simulink model "finalmodel1"  (R2024b)
(part 5 of 9)

POWER CORP D6P285A4F | NEO SOLAR POWER CORP D6P285A4FME | NEO SOLAR POWER CORP D6P285B4A | NEO SOLAR POWER CORP D6P285B4AME | NEO SOLAR POWER CORP D6Q285B4A | NEO SOLAR POWER CORP D6Q285B4AME | NEO SOLAR POWER CORP 7C00-6C290 | NEO SOLAR POWER CORP 7C00-6C290-B | NEO SOLAR POWER CORP 7E00-6C290 | NEO SOLAR POWER CORP 7E00-6C290-B | NEO SOLAR POWER CORP D6M290B3A | NEO SOLAR POWER CORP D6M290B3AME | NEO SOLAR POWER CORP D6M290B4A | NEO SOLAR POWER CORP D6M290B4AME | NEO SOLAR POWER CORP D6M290E3A | NEO SOLAR POWER CORP D6M290H3A | NEO SOLAR POWER CORP D6P290A4F | NEO SOLAR POWER CORP D6P290A4FME | NEO SOLAR POWER CORP D6P290B4A | NEO SOLAR POWER CORP D6P290B4AME | NEO SOLAR POWER CORP D6Q290B4A | NEO SOLAR POWER CORP D6Q290B4AME | NEO SOLAR POWER CORP 7C00-6C295 | NEO SOLAR POWER CORP 7C00-6C295-B | NEO SOLAR POWER CORP 7E00-6C295 | NEO SOLAR POWER CORP 7E00-6C295-B | NEO SOLAR POWER CORP D6M295B3A | NEO SOLAR POWER CORP D6M295B3AME | NEO SOLAR POWER CORP D6M295B4A | NEO SOLAR POWER CORP D6M295B4AME | NEO SOLAR POWER CORP D6M295E3A | NEO SOLAR POWER CORP D6M295H3A | NEO SOLAR POWER CORP D6P295B4A | NEO SOLAR POWER CORP D6P295B4AME | NEO SOLAR POWER CORP D6Q295B4A | NEO SOLAR POWER CORP D6Q295B4AME | NEO SOLAR POWER CORP 7E00-6C300 | NEO SOLAR POWER CORP 7E00-6C300-B | NEO SOLAR POWER CORP D6M300B3A | NEO SOLAR POWER CORP D6M300B3AME | NEO SOLAR POWER CORP D6M300B4A | NEO SOLAR POWER CORP D6M300B4AME | NEO SOLAR POWER CORP D6M300E3A | NEO SOLAR POWER CORP D6M300H3A | NEO SOLAR POWER CORP D6P300B4A | NEO SOLAR POWER CORP D6P300B4AME | NEO SOLAR POWER CORP 7E00-6C305 | NEO SOLAR POWER CORP 7E00-6C305-B | NEO SOLAR POWER CORP D6M305B4A | NEO SOLAR POWER CORP D6M305B4AME | NEO SOLAR POWER CORP D6M305E3A | NEO SOLAR POWER CORP D6M305H3A | NEO SOLAR POWER CORP D6P305B4A | NEO SOLAR POWER CORP D6P305B4AME | NEO SOLAR POWER CORP D6M310B4A | NEO SOLAR POWER CORP D6M310B4AME | NEO SOLAR POWER CORP D6M310E3A | NEO SOLAR POWER CORP D6M310H3A | NEO SOLAR POWER CORP D6P310B4A | NEO SOLAR POWER CORP D6P310B4AME | NEO SOLAR POWER CORP D6M315B4A | NEO SOLAR POWER CORP D6M315B4AME | NEO SOLAR POWER CORP D6M315E4A | NEO SOLAR POWER CORP D6M315E4AME | NEO SOLAR POWER CORP D6M315H3A | NEO SOLAR POWER CORP D6P315B4A | NEO SOLAR POWER CORP D6P315B4AME | NEO SOLAR POWER CORP D6M320B4A | NEO SOLAR POWER CORP D6M320B4AME | NEO SOLAR POWER CORP D6M320E4A | NEO SOLAR POWER CORP D6M320E4AME | NEO SOLAR POWER CORP D6M320H3A | NEO SOLAR POWER CORP D6P320B4A | NEO SOLAR POWER CORP D6P320B4AME | NEO SOLAR POWER CORP D6M325B4A | NEO SOLAR POWER CORP D6M325B4AME | NEO SOLAR POWER CORP D6M325E4A | NEO SOLAR POWER CORP D6M325E4AME | NEO SOLAR POWER CORP D6M325H3A | NEO SOLAR POWER CORP D6P325B4A | NEO SOLAR POWER CORP D6P325B4AME | NEO SOLAR POWER CORP D6M330B4A | NEO SOLAR POWER CORP D6M330B4AME | NEO SOLAR POWER CORP D6M330E4A | NEO SOLAR POWER CORP D6M330E4AME | NEO SOLAR POWER CORP D6M330H4A | NEO SOLAR POWER CORP D6P330B4A | NEO SOLAR POWER CORP D6P330B4AME | NEO SOLAR POWER CORP D6M335B4A | NEO SOLAR POWER CORP D6M335B4AME | NEO SOLAR POWER CORP D6M335E4A | NEO SOLAR POWER CORP D6M335E4AME | NEO SOLAR POWER CORP D6M335H4A | NEO SOLAR POWER CORP D6M340E4A | NEO SOLAR POWER CORP D6M340E4AME | NEO SOLAR POWER CORP D6M340H4A | NEO SOLAR POWER CORP D6M345E4A | NEO SOLAR POWER CORP D6M345E4AME | NEO SOLAR POWER CORP D6M345H4A | NEO SOLAR POWER CORP D6M350E4A | NEO SOLAR POWER CORP D6M350E4AME | NEO SOLAR POWER CORP D6M350H4A | NEO SOLAR POWER CORP D6M355E4A | NEO SOLAR POWER CORP D6M355E4AME | NEO SOLAR POWER CORP D6M355H4A | NEO SOLAR POWER CORP D6M360E4A | NEO SOLAR POWER CORP D6M360E4AME | NEO SOLAR POWER CORP D6M360H4A | NEO SOLAR POWER CORP D6M365E4A | NEO SOLAR POWER CORP D6M365E4AME | NEO SOLAR POWER CORP D6M365H4A | NEO SOLAR POWER CORP D6M370E4A | NEO SOLAR POWER CORP D6M370E4AME | NEO SOLAR POWER CORP D6M370H4A | NEO SOLAR POWER CORP D6M375E4A | NEO SOLAR POWER CORP D6M375E4AME | NEO SOLAR POWER CORP D6M375H4A | NEO SOLAR POWER CORP D6M380E4A | NEO SOLAR POWER CORP D6M380E4AME | NEO SOLAR POWER CORP D6M380H4A | NexPower Technology NH-100UT_3A | NexPower Technology NH-100UX 3A | NexPower Technology NH-100UT_4A | NexPower Technology NH-100UX 4A | NexPower Technology NH-100UT_5A | NexPower Technology NH-100UX 5A | NexPower Technology NH-100UT_6A | NexPower Technology NT-125UX | NexPower Technology NT-130UX | NexPower Technology NT-135UX | NexPower Technology NT-140UX | NexPower Technology NT-145UX | NexPower Technology NT-150 | NexPower Technology NT-155 | Next Solar Systems NXT18m | Next Solar Systems NXT20e | NICOR NS-H115M54-01 | NICOR NS-H120M54-01 | NICOR NS-H125M54-01 | NICOR NS-H160M72-01 | NICOR NS-H165M72-01 | NICOR NS-H170M72-01 | NICOR NS-H175M72-01 | NICOR NS-H180M72-01 | NICOR NS-H185M72-01 | NICOR NS-H190M72-01 | NICOR NS-H195M72-01 | NICOR NS-H200M72-01 | NICOR NS-H200P60-01 | NICOR NS-H205P60-01 | NICOR NS-H210P60-01 | NICOR NS-H215P60-01 | NICOR NS-H220P60-01 | NICOR NS-H225P60-01 | NICOR NS-H230P60-01 | NICOR NS-H235P60-01 | NICOR NS-H240P60-01 | Ningbo Best Solar Energy Technology B155(35)P1580X800 | Ningbo Best Solar Energy Technology B160(35)P1580X800 | Ningbo Best Solar Energy Technology B165(35)P1580X800 | Ningbo Best Solar Energy Technology B175(35)P1580X800 | Ningbo Best Solar Energy Technology B180(35)P1580X800 | Ningbo Maxsolar MP-150WP | Ningbo Maxsolar MP-155WP | Ningbo Maxsolar MP-160WP | Ningbo Maxsolar MP-165WP | Ningbo Maxsolar MP-170WP | Ningbo Maxsolar MP-175WP | Ningbo Maxsolar MP-180WP | Ningbo Qixin Solar Electrical Appliance SL160UL-36M | Ningbo Qixin Solar Electrical Appliance SL165UL-36M | Ningbo Qixin Solar Electrical Appliance SL170UL-36M | Ningbo Qixin Solar Electrical Appliance SL180UL-36M | Ningbo Qixin Solar Electrical Appliance SL185UL-36M | Ningbo Qixin Solar Electrical Appliance SL210UL-30P | Ningbo Qixin Solar Electrical Appliance SL215UL-30P | Ningbo Qixin Solar Electrical Appliance SL220UL-30P | Ningbo Qixin Solar Electrical Appliance SL220UL-48M | Ningbo Qixin Solar Electrical Appliance SL225UL-30P | Ningbo Qixin Solar Electrical Appliance SL225UL-48M | Ningbo Qixin Solar Electrical Appliance SL230UL-30P | Ningbo Qixin Solar Electrical Appliance SL230UL-48M | Ningbo Qixin Solar Electrical Appliance SL235UL-30P | Ningbo Qixin Solar Electrical Appliance SL235UL-48M | Ningbo Qixin Solar Electrical Appliance SL240UL-48M | Ningbo Qixin Solar Electrical Appliance SL245UL-48M | Ningbo Qixin Solar Electrical Appliance SL250UL-36M | Ningbo Qixin Solar Electrical Appliance SL250UL-48M | Ningbo Qixin Solar Electrical Appliance SL255UL-36M | Ningbo Qixin Solar Electrical Appliance SL260UL-36M | Ningbo Qixin Solar Electrical Appliance SL265UL-36M | Ningbo Qixin Solar Electrical Appliance SL270UL-36M | Ningbo Qixin Solar Electrical Appliance SL275UL-36M | Ningbo Qixin Solar Electrical Appliance SL280UL-36M | Ningbo Solar Electric Power TDB125x125-72-P 150W | Ningbo Solar Electric Power TPB125x125-72-P 150W | Ningbo Solar Electric Power TDB125x125-72-P 155W | Ningbo Solar Electric Power TPB125x125-72-P 155W | Ningbo Solar Electric Power TDB125x125-72-P 160W | Ningbo Solar Electric Power TPB125x125-72-P 160W | Ningbo Solar Electric Power TDB125x125-72-P 165W | Ningbo Solar Electric Power TPB125x125-72-P 165W | Ningbo Solar Electric Power TDB125x125-72-P 170W | Ningbo Solar Electric Power TPB125x125-72-P 170W | Ningbo Solar Electric Power TDB125x125-72-P 175W | Ningbo Solar Electric Power TPB125x125-72-P 175W | Ningbo Solar Electric Power TDB125x125-72-P 180W | Ningbo Solar Electric Power TPB125x125-72-P 180W | Ningbo Solar Electric Power TPB156x156-54-P 180W | Ningbo Solar Electric Power TPB156x156-54-P 185W | Ningbo Solar Electric Power TPB156x156-54-P 190W | Ningbo Solar Electric Power TPB156x156-54-P 195W | Ningbo Solar Electric Power TPB125x125-96-P 200W | Ningbo Solar Electric Power TPB156x156-54-P 200W | Ningbo Solar Electric Power TPB156x156-60-P 200W | Ningbo Solar Electric Power TPB156x156-60-P 205W | Ningbo Solar Electric Power TPB125x125-96-P 210W | Ningbo Solar Electric Power TPB156x156-60-P 210W | Ningbo Solar Electric Power TPB156x156-60-P 215W | Ningbo Solar Electric Power TPB125x125-96-P 220W | Ningbo Solar Electric Power TPB156x156-60-P 220W | Ningbo Solar Electric Power TPB156x156-60-P 225W | Ningbo Solar Electric Power TPB125x125-96-P 230W | Ningbo Solar Electric Power TPB156x156-60-P 230W | Ningbo Solar Electric Power TPB156x156-72-P 230W | Ningbo Solar Electric Power TPB125x125-96-P 240W | Ningbo Solar Electric Power TPB156x156-72-P 240W | Ningbo Solar Electric Power TPB156x156-72-P 250W | Ningbo Solar Electric Power TPB156x156-72-P 255W | Ningbo Solar Electric Power TPB156x156-72-P 260W | Ningbo Solar Electric Power TPB156x156-72-P 270W | Ningbo Solar Electric Power TPB156x156-72-P 280W | Ningbo Ulica Solar Science & Technology 165(35) D UL811x1581 | Ningbo Ulica Solar Science & Technology UL-180D | Ningbo Ulica Solar Science & Technology UL-185D | Ningbo Ulica Solar Science & Technology UL-190D | Ningbo Ulica Solar Science & Technology 230(35) D UL997x1953 | Ningbo Ulica Solar Science & Technology UL-230D | Ningbo Ulica Solar Science & Technology UL-230P | Ningbo Ulica Solar Science & Technology UL-235D | Ningbo Ulica Solar Science & Technology UL-235P | Ningbo Ulica Solar Science & Technology UL-240D | Ningbo Ulica Solar Science & Technology UL-240D-96 | Ningbo Ulica Solar Science & Technology UL-240P | Ningbo Ulica Solar Science & Technology UL-245D | Ningbo Ulica Solar Science & Technology UL-245D-96 | Ningbo Ulica Solar Science & Technology UL-245P | Ningbo Ulica Solar Science & Technology UL-250D | Ningbo Ulica Solar Science & Technology UL-250D-96 | Ningbo Ulica Solar Science & Technology UL-250P | Ningbo Ulica Solar Science & Technology UL-255D-96 | Ningbo Ulica Solar Science & Technology UL-260D-96 | Ningbo Ulica Solar Science & Technology UL-275D | Ningbo Ulica Solar Science & Technology UL-275P | Ningbo Ulica Solar Science & Technology UL-280D | Ningbo Ulica Solar Science & Technology UL-280P | Ningbo Ulica Solar Science & Technology UL-285D | Ningbo Ulica Solar Science & Technology UL-285P | Ningbo Ulica Solar Science & Technology UL-290D | Ningbo Ulica Solar Science & Technology UL-290P | Ningbo Ulica Solar Science & Technology UL-295D | Ningbo Ulica Solar Science & Technology UL-295P | Ningbo Ulica Solar Science & Technology UL-300D | Ningxia Yinxing Energy Photovoltaic Equipment Manufacturing YXGF-180M72 | Ningxia Yinxing Energy Photovoltaic Equipment Manufacturing YXGF-185M72 | Ningxia Yinxing Energy Photovoltaic Equipment Manufacturing YXGF-190M72 | Ningxia Yinxing Energy Photovoltaic Equipment Manufacturing YXGF-195M72 | Ningxia Yinxing Energy Photovoltaic Equipment Manufacturing YXGF-200M72 | Ningxia Yinxing Energy Photovoltaic Equipment Manufacturing YXGF-205M72 | Ningxia Yinxing Energy Photovoltaic Equipment Manufacturing YXGF-210M72 | Ningxia Yinxing Energy Photovoltaic Equipment Manufacturing YXGF-230P60 | Ningxia Yinxing Energy Photovoltaic Equipment Manufacturing YXGF-235P60 | Ningxia Yinxing Energy Photovoltaic Equipment Manufacturing YXGF-240P60 | Ningxia Yinxing Energy Photovoltaic Equipment Manufacturing YXGF-245P60 | Ningxia Yinxing Energy Photovoltaic Equipment Manufacturing YXGF-250P60 | Ningxia Yinxing Energy Photovoltaic Equipment Manufacturing YXGF-255P60 | Ningxia Yinxing Energy Photovoltaic Equipment Manufacturing YXGF-275P72 | Ningxia Yinxing Energy Photovoltaic Equipment Manufacturing YXGF-280P72 | Ningxia Yinxing Energy Photovoltaic Equipment Manufacturing YXGF-285P72 | Ningxia Yinxing Energy Photovoltaic Equipment Manufacturing YXGF-290M72 | Ningxia Yinxing Energy Photovoltaic Equipment Manufacturing YXGF-290P72 | Ningxia Yinxing Energy Photovoltaic Equipment Manufacturing YXGF-295M72 | Ningxia Yinxing Energy Photovoltaic Equipment Manufacturing YXGF-295P72 | Ningxia Yinxing Energy Photovoltaic Equipment Manufacturing YXGF-300M72 | Ningxia Yinxing Energy Photovoltaic Equipment Manufacturing YXGF-300P72 | Ningxia Yinxing Energy Photovoltaic Equipment Manufacturing YXGF-305M72 | Ningxia Yinxing Energy Photovoltaic Equipment Manufacturing YXGF-305P72 | Nu-Cell Technologies NCT250-5M812 | Nu-Cell Technologies NCT255-5M812 | Nu-Cell Technologies NCT260-5M812 | Nu-Cell Technologies NCT265-5M812 | Nu-Cell Technologies NCT270-5M812 | Nu-Cell Technologies NCT270-6M612 | Nu-Cell Technologies NCT275-6M612 | Nu-Cell Technologies NCT280-6M612 | Nu-Cell Technologies NCT285-6M612 | Nu-Cell Technologies NCT290-6M612 | Nusun Solar NS280-6M7 | NuvoSun FL0912-90 | NuvoSun FL0912-95 | NuvoSun FL0912-100 | NuvoSun FL0912-105 | NuvoSun FL0432-110 | NuvoSun FL0912-110 | NuvoSun FL0432-115 | NuvoSun FL0912-115 | NuvoSun FL0432-120 | NuvoSun FL0432-125 | NuvoSun FL0432-130 | NuvoSun FL0927-230 | NuvoSun FL0927-240 | NuvoSun FL0927-250 | NuvoSun FL0927-260 | NuvoSun FL0927-270 | NuvoSun FL0927-280 | NuvoSun FL0927-290 | NuvoSun FL1132-350 | NuvoSun FL1132-360 | NuvoSun FL1132-370 | NuvoSun FL1132-380 | NuvoSun FL1132-390 | NuvoSun FL1132-400 | NuvoSun FL1132-410 | NuvoSun FL1132-420 | NuvoSun FL1132-430 | NuvoSun FL1132-440 | Panasonic Eco Solutions Canada PE240M-BBB | Panasonic Eco Solutions Canada PE240P-BBB | Panasonic Eco Solutions Canada PE245M-BBB | Panasonic Eco Solutions Canada PE245P-BBB | Panasonic Eco Solutions Canada PE250M-BBB | Panasonic Eco Solutions Canada PE250P-BBB | Panasonic Eco Solutions Canada PE255M-BBB | Panasonic Eco Solutions Canada PE255P-BBB | Panasonic Eco Solutions Canada PE260M-BBB | Panasonic Eco Solutions Canada PE290M-BBB | Panasonic Eco Solutions Canada PE290P-BBB | Panasonic Eco Solutions Canada PE295M-BBB | Panasonic Eco Solutions Canada PE295P-BBB | Panasonic Eco Solutions Canada PE300M-BBB | Panasonic Eco Solutions Canada PE300P-BBB | Panasonic Eco Solutions Canada PE305M-BBB | Panasonic Eco Solutions Canada PE305P-BBB | Panasonic Eco Solutions Canada PE310M-BBB | Panasonic Eco Solutions Canada PE310P-BBB | Panasonic Eco Solutions Canada PE315M-BBB | Panasonic Eco Solutions Canada PE320M-BBB | PEIMAR SG160M | PEIMAR SG165M | PEIMAR SG170M | PEIMAR SG175M | PEIMAR SG180M | PEIMAR SG185M | PEIMAR SG190M | PEIMAR SG195M | PEIMAR SG200M | PEIMAR SG205P | PEIMAR SG210P | PEIMAR SG215P | PEIMAR SG220M | PEIMAR SG220P | PEIMAR SG225M | PEIMAR SG225P | PEIMAR SG230M | PEIMAR SG230P | PEIMAR SG235M | PEIMAR SG235P | PEIMAR SG240M | PEIMAR SG240P | PEIMAR SG245M | PEIMAR SG245P | PEIMAR SG250M | PEIMAR SG250P | PEIMAR SG255M | PEIMAR SG255P | PEIMAR SG255P-72 | PEIMAR SG260M | PEIMAR SG260P | PEIMAR SG260P-72 | PEIMAR SG265M | PEIMAR SG265P | PEIMAR SG265P-72 | PEIMAR OS270M | PEIMAR SG270M | PEIMAR SG270P | PEIMAR SG270P-72 | PEIMAR OS275M | PEIMAR SG275M | PEIMAR SG275P | PEIMAR SG275P-72 | PEIMAR OS280M | PEIMAR SG280M | PEIMAR SG280P | PEIMAR SG280P-72 | PEIMAR OS285M | PEIMAR SG285M | PEIMAR SG285P | PEIMAR SG285P-72 | PEIMAR OS290M | PEIMAR SG290M | PEIMAR SG290P | PEIMAR SG290P-72 | PEIMAR OS295M | PEIMAR SG295M | PEIMAR SG295P | PEIMAR SG295P-72 | PEIMAR SG300P | PEIMAR SG300P-72 | PEIMAR OS305M | PEIMAR SG305M | PEIMAR SG305P | PEIMAR SG305P-72 | PEIMAR OS310M | PEIMAR SG310M | PEIMAR SG310P | PEIMAR SG310P-72 | PEIMAR OS315M | PEIMAR SG315M | PEIMAR SG315P | PEIMAR SG315P-72 | PEIMAR OS320M | PEIMAR SG320M | PEIMAR SG320P | PEIMAR SG320P-72 | PEIMAR OS325M | PEIMAR SG325M | PEIMAR SG325P | PEIMAR SG325P-72 | PEIMAR OS330M | PEIMAR SG330M | PEIMAR SG330P | PEIMAR SG330P-72 | PEIMAR SG335M | PEIMAR SG340M | PEIMAR SG345M | PEIMAR SG350M | PEIMAR SG355M | PEIMAR SG360M | PEIMAR SG365M | PEIMAR SG370M | Perfect Source Technology PST 170 3GP48 | Perfect Source Technology PST 176 3GP48 | Perfect Source Technology PST 182 3GM48 | Perfect Source Technology PST 182 3GP48 | Perfect Source Technology PST 188 3GM48 | Perfect Source Technology PST 188 3GP48 | Perfect Source Technology PST 194 3GM48 | Perfect Source Technology PST 194 3GP48 | Perfect Source Technology PST 194 3GP54 | Perfect Source Technology PST 200 3GM48 | Perfect Source Technology PST 200 3GP48 | Perfect Source Technology PST 200 3GP54 | Perfect Source Technology PST 206 3GM48 | Perfect Source Technology PST 206 3GP54 | Perfect Source Technology PST 212 3GM48 | Perfect Source Technology PST 212 3GM54 | Perfect Source Technology PST 212 3GP54 | Perfect Source Technology PST 212GT | Perfect Source Technology PST 218 3GM54 | Perfect Source Technology PST 218 3GP54 | Perfect Source Technology PST 218 3GP60 | Perfect Source Technology PST 218GT | Perfect Source Technology PST 224 3GM54 | Perfect Source Technology PST 224 3GM60 | Perfect Source Technology PST 224 3GP60 | Perfect Source Technology PST 224GT | Perfect Source Technology PST 230 3GM54 | Perfect Source Technology PST 230 3GM60 | Perfect Source Technology PST 230 3GP60 | Perfect Source Technology PST 230GT | Perfect Source Technology PST 236 3GM54 | Perfect Source Technology PST 236 3GM60 | Perfect Source Technology PST 236 3GP60 | Perfect Source Technology PST 236GT | Perfect Source Technology PST 242 3GM60 | Perfect Source Technology PST 242 3GP60 | Perfect Source Technology PST 248 3GM60 | Perfect Source Technology PST 248 3GP60 | Perfect Source Technology PST 254 3GM60 | Perfect Source Technology PST 254 3GP60 | Perfectenergy (Shanghai) PEM-160/180-72M | Perfectenergy (Shanghai) PEM-250-60M6 | Perfectenergy (Shanghai) PEM-255-60M6 | Perfectenergy (Shanghai) PEM-260-60M6 | Perfectenergy (Shanghai) PEM-265-60M6 | Perfectenergy (Shanghai) PEM-270-60M6 | Perlight Solar PLM-175M-72 | Perlight Solar PLM-185M-72 | Perlight Solar PLM-205P-60 | Perlight Solar PLM-210P-60 | Perlight Solar PLM-215P-60 | Perlight Solar PLM-220P-60 | Perlight Solar PLM-225P-60 | Perlight Solar PLM-230P-60 | Perlight Solar PLM-235P-60 | Perlight Solar PLM-240M-60 | Perlight Solar PLM-240P-60 | Perlight Solar PLM-245M-60 | Perlight Solar PLM-250M-60 | Perlight Solar PLM-255M-60 | Perlight Solar PLM-270P-72 | Perlight Solar PLM-275P-72 | Perlight Solar PLM-280P-72 | Perlight Solar PLM-285P-72 | Perlight Solar PLM-290M-72 | Perlight Solar PLM-290P-72 | Perlight Solar PLM-295M-72 | Perlight Solar PLM-300M-72 | Perlight Solar PLM-305M-72 | Pevafersa America IP-220 GG | Pevafersa America IP-225 GG | Pevafersa America IP-230 GG | Pevafersa America IP-235 GG | Philadelphia Solar PS-M36S-90 | Philadelphia Solar PS-M36S-95 | Philadelphia Solar PS-P36-130 | Philadelphia Solar PS-P36-135 | Philadelphia Solar PS-P36-140 | Philadelphia Solar PS-P36-145 | Philadelphia Solar PS-M72S-180 | Philadelphia Solar PS-M72S-185 | Philadelphia Solar PS-M72S-190 | Philadelphia Solar PS-P54-205 | Philadelphia Solar PS-P54-210 | Philadelphia Solar PS-P54-215 | Philadelphia Solar PS-P54-220 | Philadelphia Solar PS-P60-220 | Philadelphia Solar PS-P54-225 | Philadelphia Solar PS-P60-230 | Philadelphia Solar PS-P60-235 | Philadelphia Solar PS-P60-240 | Philadelphia Solar PS-P60-245 | Philadelphia Solar PS-P60-250 | Philadelphia Solar PS-P60-255 | Philadelphia Solar PS-P60-260 | Philadelphia Solar PS-P60-265 | Philadelphia Solar PS-M60-270 | Philadelphia Solar PS-P72-270 | Philadelphia Solar PS-M60-275 | Philadelphia Solar PS-P72-275 | Philadelphia Solar PS-M60-280 | Philadelphia Solar PS-P72-280 | Philadelphia Solar PS-P72-285 | Philadelphia Solar PS-P72-290 | Philadelphia Solar PS-P72-300 | Philadelphia Solar PS-P72-305 | Philadelphia Solar PS-P72-310 | Philadelphia Solar PS-P72-315 | Phono Solar Technology PS160M-24/F | Phono Solar Technology PS165M-24/F | Phono Solar Technology PS170M-24/F | Phono Solar Technology PS180M-24/F | Phono Solar Technology PS185M-24/F | Phono Solar Technology PS190M-24/F | Phono Solar Technology PS195M-24/F | Phono Solar Technology PS200M-24/F | Phono Solar Technology PS210M-20/U | Phono Solar Technology PS210P-20/U | Phono Solar Technology PS-215M-18/VT | Phono Solar Technology PS215M-20/U | Phono Solar Technology PS215P-20/U | Phono Solar Technology PS-220M-18/VT | Phono Solar Technology PS220M-20/U | Phono Solar Technology PS-220M-20/UT | Phono Solar Technology PS220P-20/U | Phono Solar Technology PS-220P-20/UT | Phono Solar Technology PS-225M-18/VT | Phono Solar Technology PS225M-20/U | Phono Solar Technology PS-225M-20/UT | Phono Solar Technology PS225P-20/U | Phono Solar Technology PS-225P-20/UT | Phono Solar Technology PS230M-20/U | Phono Solar Technology PS-230M-20/UT | Phono Solar Technology PS230MB-20/U | Phono Solar Technology PS230P-20/U | Phono Solar Technology PS-230P-20/UT | Phono Solar Technology PS230PB-20/U | Phono Solar Technology PS235M-20/U | Phono Solar Technology PS-235M-20/UT | Phono Solar Technology PS235MB-20/U | Phono Solar Technology PS235P-20/U | Phono Solar Technology PS235PB-20/U | Phono Solar Technology PS-240M-18/VT | Phono Solar Technology PS240M-20/U | Phono Solar Technology PS240M-20/U-AC | Phono Solar Technology PS-240M-20/UT | Phono Solar Technology PS240MB-20/U | Phono Solar Technology PS240P-20/U | Phono Solar Technology PS240P-20/U-AC | Phono Solar Technology PS-240P-20/UT | Phono Solar Technology PS240PB-20/U | Phono Solar Technology PS245M | Phono Solar Technology PS245M-20/U | Phono Solar Technology PS245M-20/U-AC | Phono Solar Technology PS-245M-20/UT | Phono Solar Technology PS245MB-20/U | Phono Solar Technology PS245P-20/U | Phono Solar Technology PS245P-20/U-AC | Phono Solar Technology PS-245P-20/UT | Phono Solar Technology PS245PB-20/U | Phono Solar Technology PS 250P-20/UV | Phono Solar Technology PS250M | Phono Solar Technology PS250M-20/U | Phono Solar Technology PS250M-20/U-AC | Phono Solar Technology PS-250M-20/UT | Phono Solar Technology PS-250M-24/TT | Phono Solar Technology PS250MB-20/U | Phono Solar Technology PS250P-20/U-AC | Phono Solar Technology PS-250P-20/UT | Phono Solar Technology PS250PB-20/U | Phono Solar Technology PS 255P-20/UV | Phono Solar Technology PS255M-20/U | Phono Solar Technology PS255M-20/U-AC | Phono Solar Technology PS-255M-20/UT | Phono Solar Technology PS255MB-20/U | Phono Solar Technology PS255P-20/U-AC | Phono Solar Technology PS-255P-20/UT | Phono Solar Technology PS255PB-20/U | Phono Solar Technology PS 260M-20/UV | Phono Solar Technology PS 260P-20/UV | Phono Solar Technology PS260M-20/U-AC | Phono Solar Technology PS-260M-20/UT | Phono Solar Technology PS260M-24/T | Phono Solar Technology PS260MB-20/U | Phono Solar Technology PS260P-20/U-AC | Phono Solar Technology PS-260P-20/UT | Phono Solar Technology PS260P-24/T | Phono Solar Technology PS260PB-20/U | Phono Solar Technology PS 265M-20/UV | Phono Solar Technology PS 265P-20/UV | Phono Solar Technology PS-265M-20/UT | Phono Solar Technology PS-265M-24/TT | Phono Solar Technology PS 270M-20/UV | Phono Solar Technology PS 270P-20/UV | Phono Solar Technology PS-270M-20/UT | Phono Solar Technology PS270M-24/T | Phono Solar Technology PS-270M-24/TT | Phono Solar Technology PS270P-24/T | Phono Solar Technology PS 275M-20/UV | Phono Solar Technology PS-275M-20/UT | Phono Solar Technology PS-275M-24/TT | Phono Solar Technology PS-275P-24/TT | Phono Solar Technology PS 280M-20/UV | Phono Solar Technology PS-280M-20/UT | Phono Solar Technology PS280M-24/T | Phono Solar Technology PS-280M-24/TT | Phono Solar Technology PS280MB-24/T | Phono Solar Technology PS280P-24/T | Phono Solar Technology PS-280P-24/TT | Phono Solar Technology PS280PB-24/T | Phono Solar Technology PS285M-24/T | Phono Solar Technology PS-285M-24/TT | Phono Solar Technology PS285MB-24/T | Phono Solar Technology PS285P-24/T | Phono Solar Technology PS-285P-24/TT | Phono Solar Technology PS285PB-24/T | Phono Solar Technology PS290M-24/T | Phono Solar Technology PS-290M-24/TT | Phono Solar Technology PS290MB-24/T | Phono Solar Technology PS290P-24/T | Phono Solar Technology PS-290P-24/TT | Phono Solar Technology PS290PB-24/T | Phono Solar Technology PS295M-24/T | Phono Solar Technology PS-295M-24/TT | Phono Solar Technology PS295MB-24/T | Phono Solar Technology PS-295P-24/TT | Phono Solar Technology PS295PB-24/T | Phono Solar Technology PS 300P-24/TV | Phono Solar Technology PS300M-24/T | Phono Solar Technology PS-300M-24/TT | Phono Solar Technology PS300MB-24/T | Phono Solar Technology PS-300P-24/TT | Phono Solar Technology PS300PB-24/T | Phono Solar Technology PS 305P-24/TV | Phono Solar Technology PS305M-24/T | Phono Solar Technology PS-305M-24/TT | Phono Solar Technology PS305MB-24/T | Phono Solar Technology PS-305P-24/TT | Phono Solar Technology PS305PB-24/T | Phono Solar Technology PS 310M-24/TV | Phono Solar Technology PS 310P-24/TV | Phono Solar Technology PS310M-24/T | Phono Solar Technology PS-310M-24/TT | Phono Solar Technology PS310MB-24/T | Phono Solar Technology PS-310P-24/TT | Phono Solar Technology PS310PB-24/T | Phono Solar Technology PS 315M-24/TV | Phono Solar Technology PS 315P-24/TV | Phono Solar Technology PS-315M-24/TT | Phono Solar Technology PS315MB-24/T | Phono Solar Technology PS-315P-24/TT | Phono Solar Technology PS315PB-24/T | Phono Solar Technology PS 320M-24/TV | Phono Solar Technology PS 320P-24/TV | Phono Solar Technology PS-320M-24/TT | Phono Solar Technology PS320MB-24/T | Phono Solar Technology PS320PB-24/T | Phono Solar Technology PS 325M-24/TV | Phono Solar Technology PS 325P-24/TV | Phono Solar Technology PS-325M-24/TT | Phono Solar Technology PS 330M-24/TV | Phono Solar Technology PS-330M-24/TT | Phono Solar Technology PS 335M-24/TV | Phono Solar Technology Co._ Ltd. PS250P-20/U | Phono Solar Technology Co._ Ltd. PS255P-20/U | Phono Solar Technology Co._ Ltd. PS260M-20/U | Phono Solar Technology Co._ Ltd. PS260P-20/U | Phono Solar Technology Co._ Ltd. PS265M-20/U | Phono Solar Technology Co._ Ltd. PS265P-20/U | Phono Solar Technology Co._ Ltd. PS270M-20/U | Phono Solar Technology Co._ Ltd. PS270P-20/U | Phono Solar Technology Co._ Ltd. PS275M-20/U | Phono Solar Technology Co._ Ltd. PS275P-20/U | Phono Solar Technology Co._ Ltd. PS280M-20/U | Phono Solar Technology Co._ Ltd. PS280M-20/UK | Phono Solar Technology Co._ Ltd. PS280P-20/U | Phono Solar Technology Co._ Ltd. PS285M-20/U | Phono Solar Technology Co._ Ltd. PS285M-20/UK | Phono Solar Technology Co._ Ltd. PS285P-20/U | Phono Solar Technology Co._ Ltd. PS290M-20/U | Phono Solar Technology Co._ Ltd. PS290M-20/UK | Phono Solar Technology Co._ Ltd. PS295M-20/U | Phono Solar Technology Co._ Ltd. PS295M-20/UK | Phono Solar Technology Co._ Ltd. PS295P-24/T | Phono Solar Technology Co._ Ltd. PS300M-20/UK | Phono Solar Technology Co._ Ltd. PS300P-24/T | Phono Solar Technology Co._ Ltd. PS305P-24/T | Phono Solar Technology Co._ Ltd. PS310P-24/T | Phono Solar Technology Co._ Ltd. PS315M-24/T | Phono Solar Technology Co._ Ltd. PS315P-24/T | Phono Solar Technology Co._ Ltd. PS320M-24/T | Phono Solar Technology Co._ Ltd. PS320P-24/T | Phono Solar Technology Co._ Ltd. PS320P-24/TK | Phono Solar Technology Co._ Ltd. PS325M-24/T | Phono Solar Technology Co._ Ltd. PS325P-24/T | Phono Solar Technology Co._ Ltd. PS325P-24/TK | Phono Solar Technology Co._ Ltd. PS330M-24/T | Phono Solar Technology Co._ Ltd. PS330M-24/TK | Phono Solar Technology Co._ Ltd. PS330P-24/T | Phono Solar Technology Co._ Ltd. PS330P-24/TK | Phono Solar Technology Co._ Ltd. PS335M-24/T | Phono Solar Technology Co._ Ltd. PS335M-24/TK | Phono Solar Technology Co._ Ltd. PS335P-24/T | Phono Solar Technology Co._ Ltd. PS335P-24/TK | Phono Solar Technology Co._ Ltd. PS340M-24/T | Phono Solar Technology Co._ Ltd. PS340M-24/TK | Phono Solar Technology Co._ Ltd. PS340P-24/T | Phono Solar Technology Co._ Ltd. PS340P-24/TK | Phono Solar Technology Co._ Ltd. PS345M-24/T | Phono Solar Technology Co._ Ltd. PS345M-24/TK | Phono Solar Technology Co._ Ltd. PS350M-24/T | Phono Solar Technology Co._ Ltd. PS350M-24/TK | Phono Solar Technology Co._ Ltd. PS355M-24/T | Phono Solar Technology Co._ Ltd. PS355M-24/TK | Phono Solar Technology Co._ Ltd. PS360M-24/T | Phono Solar Technology Co._ Ltd. PS360M-24/TK | Photowatt Ontario PW2300-220 | Photowatt Ontario PW2300-225 | Photowatt Ontario PW2300-230 | Photowatt Ontario PW2300-235 | Photowatt Ontario PW2300-240 | Photowatt Ontario PW2300-245 | Photowatt Ontario PW2300-250 | Photowatt Ontario PW2300-255 | Photowatt Ontario PW2750-265 | Photowatt Ontario PW2750-270 | Photowatt Ontario PW2750-275 | Photowatt Ontario PW2750-280 | Photowatt Ontario PW2750-285 | Polar Photovoltaics TFSM-T-0 | Polar Photovoltaics TFSM-T-0X | Polar Photovoltaics TFSM-T-1 | Polar Photovoltaics TFSM-T-1X | Polar Photovoltaics TFSM-T-2 | Polar Photovoltaics TFSM-T-2X | Polar Photovoltaics TFSM-T-3 | Polar Photovoltaics TFSM-T-3X | Polar Photovoltaics TFSM-T-4 | Polar Photovoltaics TFSM-T-4X | Polar Photovoltaics TFSM-T-5 | Polar Photovoltaics TFSM-T-5X | Powercom PPV-115M6 | Powercom PPV-115S6 | Powercom PPV-120M6 | Powercom PPV-120S6 | Powercom PPV-125M6 | Powercom PPV-125S6 | Powercom PPV-130M6L | Powercom PPV-140M6 | Powercom PPV-145M6 | Powercom PPV-145S6 | Powercom PPV-150M6 | Powercom PPV-150S6 | Powercom PPV-155M6 | Powercom PPV-155S6 | Powercom PPV-175M6 | Powercom PPV-180M6L | Powercom PPV-180M6 | Powercom PPV-180S6 | Powercom PPV-185M6 | Powercom PPV-185S6 | Powercom PPV-190M6 | Powercom PPV-190S6 | Powercom PPV-195M6 | Powercom PPV-200M6 | Powercom PPV-205M6 | Powercom PPV-210M6 | Powercom PPV-210M6L | Powercom PPV-215M6 | Powercom PPV-220M6 | Powercom PPV-220M6L | Powercom PPV-230M6L | Powercom PPV-225M6 | Powercom PPV-225S6 | Powercom PPV-230M6 | Powercom PPV-230S6 | Powercom PPV-235M6 | Powercom PPV-235S6 | Powercom PPV-240M6 | Powercom PPV-260M6 | Powercom PPV-260S6 | Powercom PPV-265M6 | Powercom PPV-265S6 | Powercom PPV-270M6 | Powercom PPV-270S6 | Powercom PPV-275M6 | Powercom PPV-275S6 | Powercom PPV-285S6 | Powercom PPV-290S6 | Prism Solar Technologies B 145 | Prism Solar Technologies B 150 | Prism Solar Technologies B 155 | Prism Solar Technologies B 165S | Prism Solar Technologies HB 180 | Prism Solar Technologies B 195 | Prism Solar Technologies B 200 | Prism Solar Technologies B 205 | Prism Solar Technologies Bi48-260BSTC | Prism Solar Technologies B 210 | Prism Solar Technologies Bi48-267BSTC | Prism Solar Technologies Bi48-273BSTC | Prism Solar Technologies Bi48-279BSTC | Prism Solar Technologies Bi48-286BSTC | Prism Solar Technologies B 235 | Prism Solar Technologies B 240 | Prism Solar Technologies B 245 | Prism Solar Technologies B 250 | Prism Solar Technologies B 255 | Prism Solar Technologies B260 | Prism Solar Technologies B260L | Prism Solar Technologies Bi60-330BSTC | Prism Solar Technologies Bi60S-330BSTC | Prism Solar Technologies B265 | Prism Solar Technologies B265L | Prism Solar Technologies Bi60-337BSTC | Prism Solar Technologies Bi60S-337BSTC | Prism Solar Technologies Bi60-343BSTC | Prism Solar Technologies Bi60S-343BSTC | Prism Solar Technologies Bi60-349BSTC | Prism Solar Technologies Bi60S-349BSTC | Prism Solar Technologies Bi60-356BSTC | Prism Solar Technologies Bi60S-356BSTC | Prism Solar Technologies Bi60-362BSTC | Prism Solar Technologies Bi60-368BSTC | Prism Solar Technologies Bi60-375BSTC | Prism Solar Technologies Bi72-419BSTC | Prism Solar Technologies Bi72-425BSTC | Prism Solar Technologies Bi72-432BSTC | Prism Solar Technologies Bi72-438BSTC | Prism Solar Technologies Bi72-445BSTC | Prism Solar Technologies Bi72-451BSTC | Prism Solar Technologies Bi72-457BSTC | Prism Solar Technologies_ Inc. P72-345-WB15 | Prism Solar Technologies_ Inc. P72-350-WB15 | Prism Solar Technologies_ Inc. P72-355-WB15 | Prism Solar Technologies_ Inc. P72-360-WB15 | Prism Solar Technologies_ Inc. P72-365-WB15 | Pythagoras Solar Midi PVGU Window | Pythagoras Solar Large PVGU Window | Q-Cells Q.Smart UF-70 | Q-Cells Q.Smart-70 | Q-Cells Q.Smart UF-80 | Q-Cells Q.Smart-80 | Q-Cells Q.Smart UF-85 | Q-Cells Q.Smart-85 | Q-Cells Q.Smart UF-90 | Q-Cells Q.Smart UFL-90 | Q-Cells Q.Smart-90 | Q-Cells Q.Smart UF-95 | Q-Cells Q.Smart UFL-95 | Q-Cells Q.Smart-95 | Q-Cells Q.Smart UFL-100 | Q-Cells Q.Smart UFL-105 | Q-Cells Q.Smart UFL-110 | Q-Cells Q.Smart UFL-115 | Q-Cells QC-C05-215 | Q-Cells QC-C05-220 | Q-Cells QC-C05-225 | Q-Cells Q.Base G2 230 | Q-Cells QC-C05-230 | Q-Cells Q.Base G2 235 | Q-Cells Q.Pro G2 235 | Q-Cells QC-C05-235 | Q-Cells Q.Base G2 240 | Q-Cells Q.Pro G2 240 | Q-Cells QC-C05-240 | Q-Cells Q.Base G2 245 | Q-Cells Q.Pro G2 245 | Q-Cells QC-C05-245 | Q-Cells Q.Base G2 250 | Q-Cells Q.Pro G2 250 | Q-Cells North America Q.Peak 245 | Q-Cells North America Q.Peak BLK 245 | Q-Cells North America Q.Peak 250 | Q-Cells North America Q.Peak BLK 250 | Q-Cells North America Q.Peak 255 | Q-Cells North America Q.Peak BLK 255 | Q-Cells North America Q.Peak 260 | Q-Cells North America Q.Peak 265 | Quantum Technologies QS 215W/60-156 AP 2BB | Quantum Technologies QS 220W/60-156 AP 2BB | Quantum Technologies QS 220W/60-156 SP 2BB | Quantum Technologies QS 225W/60-156 AP 2BB | Quantum Technologies QS 225W/60-156 SP 2BB | Quantum Technologies QS 225W/60-256 EM 3BB | Quantum Technologies QS 230W/60-156 SP 2BB | Realforce Power RF-215P60 | Realforce Power RF-220P60 | Realforce Power RF-225P60 | Realforce Power RF-230P60 | Realforce Power RF-235P60 | Realforce Power RF-240P60 | Realforce Power RF-245P60 | Realforce Power RF-250P60 | Realforce Power RF-255P72 | Realforce Power RF-260P72 | Realforce Power RF-265P72 | Realforce Power RF-270P72 | Realforce Power RF-275P72 | Realforce Power RF-280P72 | Realforce Power RF-285P72 | Realforce Power RF-290P72 | Realforce Power RF-295P72 | REC ScanModule SCM205 | REC ScanModule SCM210 | REC ScanModule SCM215 | REC ScanModule SCM220 | REC ScanModule SCM225 | REC Solar REC205AE-US | REC Solar REC205AE-US (BLK) | REC Solar REC205PE | REC Solar REC205PE (BLK) | REC Solar REC205PE Q2 | REC Solar REC205PE Q3 | REC Solar REC205PE-US | REC Solar REC205PE-US (BLK) | REC Solar REC210AE-US | REC Solar REC210AE-US (BLK) | REC Solar REC210PE | REC Solar REC210PE (BLK) | REC Solar REC210PE Q2 | REC Solar REC210PE Q3 | REC Solar REC210PE-US | REC Solar REC210PE-US (BLK) | REC Solar REC215AE-US | REC Solar REC215AE-US (BLK) | REC Solar REC215PE | REC Solar REC215PE (BLK) | REC Solar REC215PE2 | REC Solar REC215PE2 BLK | REC Solar REC215PE2 BLK Q2 | REC Solar REC215PE2 BLK Q3 | REC Solar REC215PE2 Q2 | REC Solar REC215PE2 Q3 | REC Solar REC215PE-US | REC Solar REC215PE-US (BLK) | REC Solar REC220AE-US | REC Solar REC220AE-US (BLK) | REC Solar REC220PE | REC Solar REC220PE (BLK) | REC Solar REC220PE2 | REC Solar REC220PE2 BLK | REC Solar REC220PE2 BLK Q2 | REC Solar REC220PE2 BLK Q3 | REC Solar REC220PE2 Q2 | REC Solar REC220PE2 Q3 | REC Solar REC220PE-US | REC Solar REC220PE-US (BLK) | REC Solar REC225AE-US | REC Solar REC225AE-US (BLK) | REC Solar REC225PE | REC Solar REC225PE (BLK) | REC Solar REC225PE2 | REC Solar REC225PE2 BLK | REC Solar REC225PE2 BLK Q2 | REC Solar REC225PE2 BLK Q3 | REC Solar REC225PE2 Q2 | REC Solar REC225PE2 Q3 | REC Solar REC225PE-US | REC Solar REC225PE-US (BLK) | REC Solar REC230AE-US | REC Solar REC230AE-US (BLK) | REC Solar REC230PE | REC Solar REC230PE (BLK) | REC Solar REC230PE2 | REC Solar REC230PE2 BLK | REC Solar REC230PE2 BLK Q2 | REC Solar REC230PE2 BLK Q3 | REC Solar REC230PE2 Q2 | REC Solar REC230PE2 Q3 | REC Solar REC230PE-US | REC Solar REC230PE-US (BLK) | REC Solar REC235PE | REC Solar REC235PE (BLK) | REC Solar REC235PE ECO | REC Solar REC235PE Q2 | REC Solar REC235PE Q2 ECO | REC Solar REC235PE Q3 | REC Solar REC235PE Q3 ECO | REC Solar REC235PE(BLK) ECO | REC Solar REC235PE2 | REC Solar REC235PE2 BLK | REC Solar REC235PE2 BLK Q2 | REC Solar REC235PE2 BLK Q3 | REC Solar REC235PE2 Q2 | REC Solar REC235PE2 Q3 | REC Solar REC235PE-US | REC Solar REC235PE-US (BLK) | REC Solar REC235PE-US ECO | REC Solar REC235PE-US(BLK) ECO | REC Solar REC240PE | REC Solar REC240PE (BLK) | REC Solar REC240PE ECO | REC Solar REC240PE Q2 | REC Solar REC240PE Q2 ECO | REC Solar REC240PE Q3 | REC Solar REC240PE Q3 ECO | REC Solar REC240PE(BLK) ECO | REC Solar REC240PE2 | REC Solar REC240PE2 BLK | REC Solar REC240PE2 BLK Q2 | REC Solar REC240PE2 BLK Q3 | REC Solar REC240PE2 Q2 | REC Solar REC240PE2 Q3 | REC Solar REC240PE-US | REC Solar REC240PE-US (BLK) | REC Solar REC240PE-US ECO | REC Solar REC240PE-US(BLK) ECO | REC Solar REC245PE | REC Solar REC245PE (BLK) | REC Solar REC245PE ECO | REC Solar REC245PE Q2 | REC Solar REC245PE Q2 ECO | REC Solar REC245PE Q3 | REC Solar REC245PE Q3 ECO | REC Solar REC245PE(BLK) ECO | REC Solar REC245PE2 | REC Solar REC245PE2 BLK | REC Solar REC245PE2 BLK Q2 | REC Solar REC245PE2 BLK Q3 | REC Solar REC245PE2 Q2 | REC Solar REC245PE2 Q3 | REC Solar REC245PE-US | REC Solar REC245PE-US (BLK) | REC Solar REC245PE-US ECO | REC Solar REC245PE-US(BLK) ECO | REC Solar REC250PE | REC Solar REC250PE (BLK) | REC Solar REC250PE BLK2 | REC Solar REC250PE BLK2 Q2 | REC Solar REC250PE BLK2 Q3 | REC Solar REC250PE ECO | REC Solar REC250PE Q2 | REC Solar REC250PE Q2 ECO | REC Solar REC250PE Q3 | REC Solar REC250PE Q3 ECO | REC Solar REC250PE Z-LINK | REC Solar REC250PE Z-Link-S | REC Solar REC250PE Z-Link-S Q2 | REC Solar REC250PE Z-Link-S Q3 | REC Solar REC250PE(BLK) ECO | REC Solar REC250PE2 | REC Solar REC250PE2 BLK | REC Solar REC250PE2 BLK Q2 | REC Solar REC250PE2 BLK Q3 | REC Solar REC250PE2 Q2 | REC Solar REC250PE2 Q3 | REC Solar REC250PE-US | REC Solar REC250PE-US (BLK) | REC Solar REC250PE-US ECO | REC Solar REC250PE-US(BLK) ECO | REC Solar REC255PE | REC Solar REC255PE BLK2 | REC Solar REC255PE BLK2 Q2 | REC Solar REC255PE BLK2 Q3 | REC Solar REC255PE Q2 | REC Solar REC255PE Q3 | REC Solar REC255PE Z-LINK | REC Solar REC255PE Z-Link-S | REC Solar REC255PE Z-Link-S Q2 | REC Solar REC255PE Z-Link-S Q3 | REC Solar REC255PE(BLK) | REC Solar REC255PE2 | REC Solar REC255PE2 BLK | REC Solar REC255PE2 BLK Q2 | REC Solar REC255PE2 BLK Q3 | REC Solar REC255PE2 Q2 | REC Solar REC255PE2 Q3 | REC Solar REC255PE-US | REC Solar REC255PE-US(BLK) | REC Solar REC260PE | REC Solar REC260PE BLK2 | REC Solar REC260PE BLK2 Q2 | REC Solar REC260PE BLK2 Q3 | REC Solar REC260PE Q2 | REC Solar REC260PE Q3 | REC Solar REC260PE Z-LINK | REC Solar REC260PE Z-Link-S | REC Solar REC260PE Z-Link-S Q2 | REC Solar REC260PE Z-Link-S Q3 | REC Solar REC260PE(BLK) | REC Solar REC260PE2 | REC Solar REC260PE2 BLK | REC Solar REC260PE2 BLK Q2 | REC Solar REC260PE2 BLK Q3 | REC Solar REC260PE2 Q2 | REC Solar REC260PE2 Q3 | REC Solar REC260PE-US | REC Solar REC260PE-US(BLK) | REC Solar REC260TP BLK | REC Solar REC260TP BLK Q2 | REC Solar REC260TP BLK Q3 | REC Solar REC260TP BLK2 | REC Solar REC260TP BLK2 Q2 | REC Solar REC260TP BLK2 Q3 | REC Solar REC265PE | REC Solar REC265PE (BLK) | REC Solar REC265PE BLK2 | REC Solar REC265PE BLK2 Q2 | REC Solar REC265PE BLK2 Q3 | REC Solar REC265PE Q2 | REC Solar REC265PE Q3 | REC Solar REC265PE Z-LINK | REC Solar REC265PE Z-Link-S | REC Solar REC265PE Z-Link-S Q2 | REC Solar REC265PE Z-Link-S Q3 | REC Solar REC265PE2 | REC Solar REC265PE2 BLK | REC Solar REC265PE2 BLK Q2 | REC Solar REC265PE2 BLK Q3 | REC Solar REC265PE2 Q2 | REC Solar REC265PE2 Q3 | REC Solar REC265PE-US | REC Solar REC265PE-US (BLK) | REC Solar REC265TP | REC Solar REC265TP BLK | REC Solar REC265TP BLK Q2 | REC Solar REC265TP BLK Q3 | REC Solar REC265TP BLK2 | REC Solar REC265TP BLK2 Q2 | REC Solar REC265TP BLK2 Q3 | REC Solar REC265TP IQ | REC Solar REC265TP IQ BLK | REC Solar REC265TP Q2 | REC Solar REC265TP Q3 | REC Solar REC270PE | REC Solar REC270PE (BLK) | REC Solar REC270PE Q2 | REC Solar REC270PE Q3 | REC Solar REC270PE Z-LINK | REC Solar REC270PE Z-Link-M | REC Solar REC270PE Z-Link-S | REC Solar REC270PE Z-Link-S Q2 | REC Solar REC270PE Z-Link-S Q3 | REC Solar REC270PE2 | REC Solar REC270PE2 BLK | REC Solar REC270PE2 BLK Q2 | REC Solar REC270PE2 BLK Q3 | REC Solar REC270PE2 Q2 | REC Solar REC270PE2 Q3 | REC Solar REC270PE-US | REC Solar REC270PE-US (BLK) | REC Solar REC270TP | REC Solar REC270TP BLK | REC Solar REC270TP BLK Q2 | REC Solar REC270TP BLK Q3 | REC Solar REC270TP BLK2 | REC Solar REC270TP BLK2 Q2 | REC Solar REC270TP BLK2 Q3 | REC Solar REC270TP IQ | REC Solar REC270TP IQ BLK | REC Solar REC270TP Q2 | REC Solar REC270TP Q3 | REC Solar REC270TP2 | REC Solar REC270TP2 BLK | REC Solar REC270TP2 BLK Q2 | REC Solar REC270TP2 BLK Q3 | REC Solar REC270TP2 BLK2 | REC Solar REC270TP2 BLK2 Q2 | REC Solar REC270TP2 BLK2 Q3 | REC Solar REC270TP2 Q2 | REC Solar REC270TP2 Q3 | REC Solar REC270TP2M BLK2 | REC Solar REC275PE Z-Link-M | REC Solar REC275TP | REC Solar REC275TP BLK | REC Solar REC275TP BLK Q2 | REC Solar REC275TP BLK Q3 | REC Solar REC275TP BLK2 | REC Solar REC275TP BLK2 Q2 | REC Solar REC275TP BLK2 Q3 | REC Solar REC275TP IQ | REC Solar REC275TP IQ BLK | REC Solar REC275TP Q2 | REC Solar REC275TP Q3 | REC Solar REC275TP2 | REC Solar REC275TP2 BLK | REC Solar REC275TP2 BLK Q2 | REC Solar REC275TP2 BLK Q3 | REC Solar REC275TP2 BLK2 | REC Solar REC275TP2 BLK2 Q2 | REC Solar REC275TP2 BLK2 Q3 | REC Solar REC275TP2 Q2 | REC Solar REC275TP2 Q3 | REC Solar REC275TP2M BLK2 | REC Solar REC280PE Z-Link-M | REC Solar REC280TP | REC Solar REC280TP BLK | REC Solar REC280TP BLK Q2 | REC Solar REC280TP BLK Q3 | REC Solar REC280TP BLK2 | REC Solar REC280TP BLK2 Q2 | REC Solar REC280TP BLK2 Q3 | REC Solar REC280TP IQ | REC Solar REC280TP IQ BLK | REC Solar REC280TP Q2 | REC Solar REC280TP Q3 | REC Solar REC280TP2 | REC Solar REC280TP2 BLK | REC Solar REC280TP2 BLK Q2 | REC Solar REC280TP2 BLK Q3 | REC Solar REC280TP2 BLK2 | REC Solar REC280TP2 BLK2 Q2 | REC Solar REC280TP2 BLK2 Q3 | REC Solar REC280TP2 Q2 | REC Solar REC280TP2 Q3 | REC Solar REC280TP2M BLK2 | REC Solar REC285PE Z-Link-M | REC Solar REC285PE72 | REC Solar REC285PE72 BLK | REC Solar REC285PE72 Q2 | REC Solar REC285PE72 Q3 | REC Solar REC285TP | REC Solar REC285TP BLK | REC Solar REC285TP BLK Q2 | REC Solar REC285TP BLK Q3 | REC Solar REC285TP IQ | REC Solar REC285TP IQ BLK | REC Solar REC285TP Q2 | REC Solar REC285TP Q3 | REC Solar REC285TP2 | REC Solar REC285TP2 BLK | REC Solar REC285TP2 BLK Q2 | REC Solar REC285TP2 BLK Q3 | REC Solar REC285TP2 BLK2 | REC Solar REC285TP2 BLK2 Q2 | REC Solar REC285TP2 BLK2 Q3 | REC Solar REC285TP2 Q2 | REC Solar REC285TP2 Q3 | REC Solar REC285TP2M BLK2 | REC Solar REC290PE Z-Link-M | REC Solar REC290PE72 | REC Solar REC290PE72 BLK | REC Solar REC290PE72 Q2 | REC Solar REC290PE72 Q3 | REC Solar REC290TP | REC Solar REC290TP BLK | REC Solar REC290TP BLK Q2 | REC Solar REC290TP BLK Q3 | REC Solar REC290TP IQ | REC Solar REC290TP IQ BLK | REC Solar REC290TP Q2 | REC Solar REC290TP Q3 | REC Solar REC290TP2 | REC Solar REC290TP2 BLK | REC Solar REC290TP2 BLK Q2 | REC Solar REC290TP2 BLK Q3 | REC Solar REC290TP2 BLK2 | REC Solar REC290TP2 BLK2 Q2 | REC Solar REC290TP2 BLK2 Q3 | REC Solar REC290TP2 Q2 | REC Solar REC290TP2 Q3 | REC Solar REC290TP2M BLK2 | REC Solar REC290TP2SM | REC Solar REC290TP2SM BLK | REC Solar REC290TP2SM BLK2 | REC Solar REC295PE72 | REC Solar REC295PE72 BLK | REC Solar REC295PE72 BLK Q2 | REC Solar REC295PE72 BLK Q3 | REC Solar REC295PE72 Q2 | REC Solar REC295PE72 Q3 | REC Solar REC295PE72XV | REC Solar REC295PE72XV Q2 | REC Solar REC295PE72XV Q3 | REC Solar REC295TP2 | REC Solar REC295TP2 Q2 | REC Solar REC295TP2 Q3 | REC Solar REC295TP2SM | REC Solar REC295TP2SM BLK | REC Solar REC295TP2SM BLK2 | REC Solar REC300PE72 | REC Solar REC300PE72 BLK | REC Solar REC300PE72 BLK Q2 | REC Solar REC300PE72 BLK Q3 | REC Solar REC300PE72 Q2 | REC Solar REC300PE72 Q3 | REC Solar REC300PE72XV | REC Solar REC300PE72XV Q2 | REC Solar REC300PE72XV Q3 | REC Solar REC300TP2 | REC Solar REC300TP2 Q2 | REC Solar REC300TP2 Q3 | REC Solar REC300TP2SM | REC Solar REC300TP2SM BLK | REC Solar REC300TP2SM BLK2 | REC Solar REC305PE72 | REC Solar REC305PE72 BLK | REC Solar REC305PE72 BLK Q2 | REC Solar REC305PE72 BLK Q3 | REC Solar REC305PE72 Q2 | REC Solar REC305PE72 Q3 | REC Solar REC305PE72XV | REC Solar REC305PE72XV Q2 | REC Solar REC305PE72XV Q3 | REC Solar REC305TP2SM | REC Solar REC305TP2SM BLK | REC Solar REC305TP2SM BLK2 | REC Solar REC310PE72 | REC Solar REC310PE72 BLK | REC Solar REC310PE72 BLK Q2 | REC Solar REC310PE72 BLK Q3 | REC Solar REC310PE72 Q2 | REC Solar REC310PE72 Q3 | REC Solar REC310PE72XV | REC Solar REC310PE72XV Q2 | REC Solar REC310PE72XV Q3 | REC Solar REC310TP2SM | REC Solar REC310TP2SM BLK | REC Solar REC310TP2SM BLK2 | REC Solar REC315PE72 | REC Solar REC315PE72 BLK | REC Solar REC315PE72 BLK Q2 | REC Solar REC315PE72 BLK Q3 | REC Solar REC315PE72 Q2 | REC Solar REC315PE72 Q3 | REC Solar REC315PE72XV | REC Solar REC315PE72XV Q2 | REC Solar REC315PE72XV Q3 | REC Solar REC315TP2SB 72 XV | REC Solar REC315TP2SM | REC Solar REC315TP2SM BLK | REC Solar REC315TP2SM BLK2 | REC Solar REC320PE72 | REC Solar REC320PE72 BLK | REC Solar REC320PE72 BLK Q2 | REC Solar REC320PE72 BLK Q3 | REC Solar REC320PE72 Q2 | REC Solar REC320PE72 Q3 | REC Solar REC320PE72XV | REC Solar REC320PE72XV Q2 | REC Solar REC320PE72XV Q3 | REC Solar REC320PEM 72 | REC Solar REC320PEM 72 BLK | REC Solar REC320PEM 72 XV | REC Solar REC320PEM 72 XV BLK | REC Solar REC320TP2SB 72 XV | REC Solar REC320TP2SM | REC Solar REC320TP2SM BLK | REC Solar REC320TP2SM BLK2 | REC Solar REC325PE72 | REC Solar REC325PE72 BLK | REC Solar REC325PE72 BLK Q2 | REC Solar REC325PE72 BLK Q3 | REC Solar REC325PE72 Q2 | REC Solar REC325PE72 Q3 | REC Solar REC325PE72XV | REC Solar REC325PE72XV Q2 | REC Solar REC325PE72XV Q3 | REC Solar REC325PEM 72 | REC Solar REC325PEM 72 BLK | REC Solar REC325PEM 72 XV | REC Solar REC325PEM 72 XV BLK | REC Solar REC325TP 72 | REC Solar REC325TP 72 BLK | REC Solar REC325TP 72 BLK Q2 | REC Solar REC325TP 72 BLK Q3 | REC Solar REC325TP 72 Q2 | REC Solar REC325TP 72 Q3 | REC Solar REC325TP 72 XV | REC Solar REC325TP 72 XV BLK | REC Solar REC325TP 72 XV BLK Q2 | REC Solar REC325TP 72 XV BLK Q3 | REC Solar REC325TP 72 XV Q2 | REC Solar REC325TP 72 XV Q3 | REC Solar REC325TP2S 72 | REC Solar REC325TP2S 72 BLK | REC Solar REC325TP2S 72 BLK2 | REC Solar REC325TP2S 72 Q2 | REC Solar REC325TP2S 72 Q3 | REC Solar REC325TP2S 72 XV | REC Solar REC325TP2S 72 XV BLK | REC Solar REC325TP2S 72 XV Q2 | REC Solar REC325TP2S 72 XV Q3 | REC Solar REC325TP2SB 72 XV | REC Solar REC330PEM 72 | REC Solar REC330PEM 72 BLK | REC Solar REC330PEM 72 XV | REC Solar REC330PEM 72 XV BLK | REC Solar REC330TP 72 | REC Solar REC330TP 72 BLK | REC Solar REC330TP 72 BLK Q2 | REC Solar REC330TP 72 BLK Q3 | REC Solar REC330TP 72 Q2 | REC Solar REC330TP 72 Q3 | REC Solar REC330TP 72 XV | REC Solar REC330TP 72 XV BLK | REC Solar REC330TP 72 XV BLK Q2 | REC Solar REC330TP 72 XV BLK Q3 | REC Solar REC330TP 72 XV Q2 | REC Solar REC330TP 72 XV Q3 | REC Solar REC330TP2S 72 | REC Solar REC330TP2S 72 BLK | REC Solar REC330TP2S 72 BLK2 | REC Solar REC330TP2S 72 Q2 | REC Solar REC330TP2S 72 Q3 | REC Solar REC330TP2S 72 XV | REC Solar REC330TP2S 72 XV BLK | REC Solar REC330TP2S 72 XV Q2 | REC Solar REC330TP2S 72 XV Q3 | REC Solar REC330TP2SB 72 XV | REC Solar REC335PEM 72 | REC Solar REC335PEM 72 BLK | REC Solar REC335PEM 72 XV | REC Solar REC335PEM 72 XV BLK | REC Solar REC335TP 72 | REC Solar REC335TP 72 BLK | REC Solar REC335TP 72 BLK Q2 | REC Solar REC335TP 72 BLK Q3 | REC Solar REC335TP 72 Q2 | REC Solar REC335TP 72 Q3 | REC Solar REC335TP 72 XV | REC Solar REC335TP 72 XV BLK | REC Solar REC335TP 72 XV BLK Q2 | REC Solar REC335TP 72 XV BLK Q3 | REC Solar REC335TP 72 XV Q2 | REC Solar REC335TP 72 XV Q3 | REC Solar REC335TP2S 72 | REC Solar REC335TP2S 72 BLK | REC Solar REC335TP2S 72 BLK2 | REC Solar REC335TP2S 72 Q2 | REC Solar REC335TP2S 72 Q3 | REC Solar REC335TP2S 72 XV | REC Solar REC335TP2S 72 XV BLK | REC Solar REC335TP2S 72 XV Q2 | REC Solar REC335TP2S 72 XV Q3 | REC Solar REC335TP2SB 72 XV | REC Solar REC340PEM 72 | REC Solar REC340PEM 72 BLK | REC Solar REC340PEM 72 XV | REC Solar REC340PEM 72 XV BLK | REC Solar REC340TP 72 | REC Solar REC340TP 72 BLK | REC Solar REC340TP 72 BLK Q2 | REC Solar REC340TP 72 BLK Q3 | REC Solar REC340TP 72 Q2 | REC Solar REC340TP 72 Q3 | REC Solar REC340TP 72 XV | REC Solar REC340TP 72 XV BLK | REC Solar REC340TP 72 XV BLK Q2 | REC Solar REC340TP 72 XV BLK Q3 | REC Solar REC340TP 72 XV Q2 | REC Solar REC340TP 72 XV Q3 | REC Solar REC340TP2S 72 | REC Solar REC340TP2S 72 BLK | REC Solar REC340TP2S 72 BLK2 | REC Solar REC340TP2S 72 Q2 | REC Solar REC340TP2S 72 Q3 | REC Solar REC340TP2S 72 XV | REC Solar REC340TP2S 72 XV BLK | REC Solar REC340TP2S 72 XV Q2 | REC Solar REC340TP2S 72 XV Q3 | REC Solar REC340TP2SB 72 XV | REC Solar REC345PEM 72 | REC Solar REC345PEM 72 BLK | REC Solar REC345PEM 72 XV | REC Solar REC345PEM 72 XV BLK | REC Solar REC345TP 72 | REC Solar REC345TP 72 BLK | REC Solar REC345TP 72 BLK Q2 | REC Solar REC345TP 72 BLK Q3 | REC Solar REC345TP 72 Q2 | REC Solar REC345TP 72 Q3 | REC Solar REC345TP 72 XV | REC Solar REC345TP 72 XV BLK | REC Solar REC345TP 72 XV BLK Q2 | REC Solar REC345TP 72 XV BLK Q3 | REC Solar REC345TP 72 XV Q2 | REC Solar REC345TP 72 XV Q3 | REC Solar REC345TP2S 72 | REC Solar REC345TP2S 72 BLK | REC Solar REC345TP2S 72 BLK2 | REC Solar REC345TP2S 72 Q2 | REC Solar REC345TP2S 72 Q3 | REC Solar REC345TP2S 72 XV | REC Solar REC345TP2S 72 XV BLK | REC Solar REC345TP2S 72 XV Q2 | REC Solar REC345TP2S 72 XV Q3 | REC Solar REC350PEM 72 | REC Solar REC350PEM 72 BLK | REC Solar REC350PEM 72 XV | REC Solar REC350PEM 72 XV BLK | REC Solar REC350TP 72 | REC Solar REC350TP 72 BLK | REC Solar REC350TP 72 BLK Q2 | REC Solar REC350TP 72 BLK Q3 | REC Solar REC350TP 72 Q2 | REC Solar REC350TP 72 Q3 | REC Solar REC350TP 72 XV | REC Solar REC350TP 72 XV BLK | REC Solar REC350TP 72 XV BLK Q2 | REC Solar REC350TP 72 XV BLK Q3 | REC Solar REC350TP 72 XV Q2 | REC Solar REC350TP 72 XV Q3 | REC Solar REC350TP2M 72 | REC Solar REC350TP2M 72 Q2 | REC Solar REC350TP2M 72 Q3 | REC Solar REC350TP2S 72 | REC Solar REC350TP2S 72 BLK | REC Solar REC350TP2S 72 BLK2 | REC Solar REC350TP2S 72 Q2 | REC Solar REC350TP2S 72 Q3 | REC Solar REC350TP2S 72 XV | REC Solar REC350TP2S 72 XV BLK | REC Solar REC350TP2S 72 XV Q2 | REC Solar REC350TP2S 72 XV Q3 | REC Solar REC350TP2SM 72 | REC Solar REC350TP2SM 72 BLK | REC Solar REC350TP2SM 72 BLK2 | REC Solar REC355PEM 72 | REC Solar REC355PEM 72 BLK | REC Solar REC355PEM 72 XV | REC Solar REC355PEM 72 XV BLK | REC Solar REC355TP 72 | REC Solar REC355TP 72 BLK | REC Solar REC355TP 72 BLK Q2 | REC Solar REC355TP 72 BLK Q3 | REC Solar REC355TP 72 Q2 | REC Solar REC355TP 72 Q3 | REC Solar REC355TP 72 XV | REC Solar REC355TP 72 XV BLK | REC Solar REC355TP 72 XV BLK Q2 | REC Solar REC355TP 72 XV BLK Q3 | REC Solar REC355TP 72 XV Q2 | REC Solar REC355TP 72 XV Q3 | REC Solar REC355TP2M 72 | REC Solar REC355TP2M 72 Q2 | REC Solar REC355TP2M 72 Q3 | REC Solar REC355TP2S 72 | REC Solar REC355TP2S 72 BLK | REC Solar REC355TP2S 72 BLK2 | REC Solar REC355TP2S 72 Q2 | REC Solar REC355TP2S 72 Q3 | REC Solar REC355TP2S 72 XV | REC Solar REC355TP2S 72 XV BLK | REC Solar REC355TP2S 72 XV Q2 | REC Solar REC355TP2S 72 XV Q3 | REC Solar REC355TP2SM 72 | REC Solar REC355TP2SM 72 BLK | REC Solar REC355TP2SM 72 BLK2 | REC Solar REC360PEM 72 | REC Solar REC360PEM 72 BLK | REC Solar REC360PEM 72 XV | REC Solar REC360PEM 72 XV BLK | REC Solar REC360TP2M 72 | REC Solar REC360TP2M 72 Q2 | REC Solar REC360TP2M 72 Q3 | REC Solar REC360TP2SM 72 | REC Solar REC360TP2SM 72 BLK | REC Solar REC360TP2SM 72 BLK2 | REC Solar REC365PEM 72 | REC Solar REC365PEM 72 BLK | REC Solar REC365PEM 72 XV | REC Solar REC365PEM 72 XV BLK | REC Solar REC365TP2M 72 | REC Solar REC365TP2M 72 Q2 | REC Solar REC365TP2M 72 Q3 | REC Solar REC365TP2SM 72 | REC Solar REC365TP2SM 72 BLK | REC Solar REC365TP2SM 72 BLK2 | REC Solar REC370PEM 72 | REC Solar REC370PEM 72 BLK | REC Solar REC370PEM 72 XV | REC Solar REC370PEM 72 XV BLK | REC Solar REC370TP2M 72 | REC Solar REC370TP2M 72 Q2 | REC Solar REC370TP2M 72 Q3 | REC Solar REC370TP2SM 72 | REC Solar REC370TP2SM 72 BLK | REC Solar REC370TP2SM 72 BLK2 | REC Solar REC375TP2M 72 | REC Solar REC375TP2M 72 Q2 | REC Solar REC375TP2M 72 Q3 | REC Solar REC375TP2SM 72 | REC Solar REC375TP2SM 72 BLK | REC Solar REC375TP2SM 72 BLK2 | REC Solar REC380TP2M 72 | REC Solar REC380TP2M 72 Q2 | REC Solar REC380TP2M 72 Q3 | REC Solar REC380TP2SM 72 | REC Solar REC380TP2SM 72 BLK | REC Solar REC380TP2SM 72 BLK2 | Recom RCM-250-6MB | Recom RCM-250-6PB | Recom RCM-255-6PB | Recom RCM-260-6MB | Recom RCM-260-6MB-BB | Recom RCM-260-6PB | Recom RCM-265-6MB-BB | Recom RCM-270-6MB | Recom RCM-270-6MB-BB | Recom RCM-275-6MB-BB | Recom RCM-280-6MB-BB | Recom RCM-285-6PA | Recom RCM-290-6PA | Recom RCM-295-6PA | Recom RCM-300-6PA | Recom RCM-305-6PA | Recom RCM-310-6PA | Recom RCM-315-6MA | Recom RCM-315-6PA | Recom RCM-320-6MA | Recom RCM-320-6PA | Recom RCM-325-6MA | Recom RCM-325-6PA | Recom RCM-330-6MA | Recom RCM-330-6PA | Recom RCM-335-6MA | Recom RCM-340-6MA | Recom RCM-345-6MA | RECOM AG RCM-285-6MB-BB | RECOM AG RCM-290-6MB-BB | RECOM AG RCM-295-6MB-BB | RECOM AG RCM-300-6MB-BB | Renesola America JC180S-24/Db | Renesola America JC185S-24/Db | Renesola America JC190S-24/Db | Renesola America JC195S-24/Db | Renesola America JC200S-24/Db | Renesola America JC220M-24/Bx | Renesola America JC225M-24/Bx | Renesola America JC225S-24/Bb | Renesola America JC230M-24/Bb | Renesola America JC230S-24/Bb | Renesola America JC235M-24/Bx | Renesola America JC235S-24/Bb | Renesola America JC240M-24/Bx | Renesola America JC240M-24/Bx-b | Renesola America JC240M-24/Bxh | Renesola America JC240M-24/Bxh-b | Renesola America JC240S-24/Bb | Renesola America JC240S-24/Bb-b | Renesola America JC245M-24/Bx | Renesola America JC245M-24/Bx-b | Renesola America JC245M-24/Bxh | Renesola America JC245M-24/Bxh-b | Renesola America JC245S-24/Bb | Renesola America JC245S-24/Bb-b | Renesola America JC250M-24/Bx | Renesola America JC250M-24/Bx-b | Renesola America JC250M-24/Bxh | Renesola America JC250M-24/Bxh-b | Renesola America JC250S-24/Bb | Renesola America JC250S-24/Bb-b | Renesola America JC250S-24/Bbh | Renesola America JC250S-24/Bbh-b | Renesola America JC255M-24/Bx | Renesola America JC255M-24/Bx-b | Renesola America JC255M-24/Bxh | Renesola America JC255M-24/Bxh-b | Renesola America JC255S-24/Bb | Renesola America JC255S-24/Bb-b | Renesola America JC255S-24/Bbh | Renesola America JC255S-24/Bbh-b | Renesola America JC260M-24/Bbs | Renesola America JC260M-24/Bbs-b | Renesola America JC260M-24/Bx | Renesola America JC260M-24/Bx-b | Renesola America JC260M-24/Bxh | Renesola America JC260M-24/Bxh-b | Renesola America JC260M-24/Bzs | Renesola America JC260M-24/Bzs-b | Renesola America JC260S-24/Bb | Renesola America JC260S-24/Bb-b | Renesola America JC265M-24/Bbs | Renesola America JC265M-24/Bbs-b | Renesola America JC265M-24/Bzs | Renesola America JC265M-24/Bzs-b | Renesola America JC265S-24/Ab | Renesola America JC270M-24/Ax | Renesola America JC270M-24/Bbs | Renesola America JC270M-24/Bbs-b | Renesola America JC270M-24/Bzs | Renesola America JC270M-24/Bzs-b | Renesola America JC270S-24/Ab | Renesola America JC275M-24/Ax | Renesola America JC275S-24/Ab | Renesola America JC280M-24/Ax | Renesola America JC280S-24/Ab | Renesola America JC285M-24/Ax | Renesola America JC285M-24/Ax-b | Renesola America JC285M-24/Axh | Renesola America JC285M-24/Axh-b | Renesola America JC285S-24/Ab | Renesola America JC290F-24/Abh-b | Renesola America JC290M-24/Ax | Renesola America JC290M-24/Ax-b | Renesola America JC290M-24/Axh | Renesola America JC290M-24/Axh-b | Renesola America JC290S-24/Ab | Renesola America JC290S-24/Abh | Renesola America JC295M-24/Abh | Renesola America JC295M-24/Abh-b | Renesola America JC295M-24/Ax | Renesola America JC295M-24/Ax-b | Renesola America JC295S-24/Ab | Renesola America JC295S-24/Abh | Renesola America JC295S-24/Abh-b | Renesola America JC300M-24/Ax | Renesola America JC300M-24/Ax-b | Renesola America JC300M-24/Axh | Renesola America JC300M-24/Axh-b | Renesola America JC300S-24/Ab | Renesola America JC300S-24/Abh | Renesola America JC300S-24/Abh-b | Renesola America JC305M-24/Ax | Renesola America JC305M-24/Ax-b | Renesola America JC305M-24/Axh | Renesola America JC305M-24/Axh-b | Renesola America JC305S-24/Abh | Renesola America JC305S-24/Abh-b | Renesola America JC310M-24/Abs | Renesola America JC310M-24/Abs-b | Renesola America JC310M-24/Ax-b | Renesola America JC310M-24/Axh | Renesola America JC310M-24/Axh-b | Renesola America JC310M-24/Azs | Renesola America JC310M-24/Azs-b | Renesola America JC310S-24/Abh | Renesola America JC310S-24/Abh-b | Renesola America JC315M-24/Abs | Renesola America JC315M-24/Abs-b | Renesola America JC315M-24/Ax-b | Renesola America JC315M-24/Axh | Renesola America JC315M-24/Axh-b | Renesola America JC315M-24/Azs | Renesola America JC315M-24/Azs-b | Renesola America JC315S-24/Abh | Renesola America JC315S-24/Abh-b | Renesola America JC320M-24/Abs | Renesola America JC320M-24/Abs-b | Renesola America JC320M-24/Azs | Renesola America JC320M-24/Azs-b | Renesola America JC320S-24/Abh | Renesola America JC320S-24/Abh-b | Renesola America JC325M-24/Abs | Renesola America JC325M-24/Abs-b | Renesola America JC325M-24/Azs | Renesola America JC325M-24/Azs-b | Renesola America JC330M-24/Abs | Renesola America JC330M-24/Abs-b | Renesola America JC330M-24/Azs | Renesola America JC330M-24/Azs-b | Renesola America JC335M-24/Abs | Renesola America JC335M-24/Abs-b | Renesola America JC335M-24/Azs | Renesola America JC335M-24/Azs-b | Renogy RNG-175D | Renogy RNG-180D | Renogy RNG-185D | Renogy RNG-215P | Renogy RNG-220P | Renogy RNG-225D | Renogy RNG-225P | Renogy RNG-230D | Renogy RNG-230P | Renogy RNG-235D | Renogy RNG-235D-60 | Renogy RNG-235P | Renogy RNG-235P-60 | Renogy RNG-240D | Renogy RNG-240D-60 | Renogy RNG-240P-60 | Renogy RNG-245D | Renogy RNG-245D-60 | Renogy RNG-245P-60 | Renogy RNG-250D-60 | Renogy RNG-250P | Renogy RNG-250P-60 | Renogy RNG-260D | Renogy RNG-260P | Renogy RNG-265D | Renogy RNG-270D | Renogy RNG-270P | Renogy RNG-275D | Renogy RNG-280D | Renogy RNG-280P | Renogy RNG-285D | Renogy RNG-285P | Renogy RNG-290D | Renogy RNG-290P | Renogy RNG-295D | Renogy RNG-295P | Renogy RNG-300D | Renogy RNG-300P | Renogy RNG-305P | Renogy RNG-310P | Renogy RNG-315P | Renogy RNG-320P | Renogy RNG-325P | Resonix EPML120W6H | Resonix EPMN120W6H | Resonix EPML130W6H | Resonix EPMN130W6H | Resonix EPML150W6H | Resonix EPMN150W6H | Resonix EPML180W6H | Resonix EPMN180W6H | Resonix EPML185W6H | Resonix EPMN185W6H | Resonix EPML220W6H | Resonix EPML225W6H | Resonix EPMN225W6H | Resonix EPML275W6H | Resonix EPMN275W6H | Risen Energy Co._ Ltd. SYP-85S | Risen Energy Co._ Ltd. SYP-110S | Risen Energy Co._ Ltd. SYP-160S | Risen Energy Co._ Ltd. SYP-165S | Risen Energy Co._ Ltd. SYP-170S | Risen Energy Co._ Ltd. SYP-175S | Risen Energy Co._ Ltd. SYP-180S | Risen Energy Co._ Ltd. SYP-185S | Risen Energy Co._ Ltd. SYP-190S | Risen Energy Co._ Ltd. SYP-195S | Risen Energy Co._ Ltd. SYP200P | Risen Energy Co._ Ltd. SYP-200S | Risen Energy Co._ Ltd. SYP-200W | Risen Energy Co._ Ltd. SYP210M | Risen Energy Co._ Ltd. SYP210P | Risen Energy Co._ Ltd. SYP-210S | Risen Energy Co._ Ltd. SYP220M | Risen Energy Co._ Ltd. SYP220P | Risen Energy Co._ Ltd. RSM60-6-230M | Risen Energy Co._ Ltd. RSM60-6-230P | Risen Energy Co._ Ltd. SYP230M | Risen Energy Co._ Ltd. SYP230P | Risen Energy Co._ Ltd. RSM60-6-235M | Risen Energy Co._ Ltd. RSM60-6-235P | Risen Energy Co._ Ltd. RSM60-6-240M | Risen Energy Co._ Ltd. RSM60-6-240P | Risen Energy Co._ Ltd. SYP240M | Risen Energy Co._ Ltd. SYP240P | Risen Energy Co._ Ltd. RSM60-6-245M | Risen Energy Co._ Ltd. RSM60-6-245P | Risen Energy Co._ Ltd. RSM60-6-250M | Risen Energy Co._ Ltd. RSM60-6-250P | Risen Energy Co._ Ltd. SYP250M | Risen Energy Co._ Ltd. SYP250P | Risen Energy Co._ Ltd. RSM60-6-255M | Risen Energy Co._ Ltd. RSM60-6-255P | Risen Energy Co._ Ltd. RSM60-6-260M | Risen Energy Co._ Ltd. RSM60-6-260P | Risen Energy Co._ Ltd. SYP260M | Risen Energy Co._ Ltd. SYP260P | Risen Energy Co._ Ltd. RSM60-6-265M | Risen Energy Co._ Ltd. RSM60-6-265P | Risen Energy Co._ Ltd. RSM60-6-270M | Risen Energy Co._ Ltd. RSM60-6-270P | Risen Energy Co._ Ltd. SYP270M | Risen Energy Co._ Ltd. SYP270P | Risen Energy Co._ Ltd. RSM60-6-275M | Risen Energy Co._ Ltd. RSM60-6-275P | Risen Energy Co._ Ltd. RSM60-6-280M | Risen Energy Co._ Ltd. RSM60-6-280P | Risen Energy Co._ Ltd. RSM72-6-280M | Risen Energy Co._ Ltd. RSM72-6-280P | Risen Energy Co._ Ltd. SYP280M | Risen Energy Co._ Ltd. SYP280P | Risen Energy Co._ Ltd. RSM60-6-285M | Risen Energy Co._ Ltd. RSM60-6-285P | Risen Energy Co._ Ltd. RSM72-6-285M | Risen Energy Co._ Ltd. RSM72-6-285P | Risen Energy Co._ Ltd. RSM60-6-290M | Risen Energy Co._ Ltd. RSM72-6-290M | Risen Energy Co._ Ltd. RSM72-6-290P | Risen Energy Co._ Ltd. SYP290M | Risen Energy Co._ Ltd. RSM72-6-295M | Risen Energy Co._ Ltd. RSM72-6-295P | Risen Energy Co._ Ltd. RSM72-6-300M | Risen Energy Co._ Ltd. RSM72-6-300P | Risen Energy Co._ Ltd. SYP300M | Risen Energy Co._ Ltd. RSM72-6-305M | Risen Energy Co._ Ltd. RSM72-6-305P | Risen Energy Co._ Ltd. SYP305M | Risen Energy Co._ Ltd. RSM72-6-310M | Risen Energy Co._ Ltd. RSM72-6-310P | Risen Energy Co._ Ltd. RSM72-6-315M | Risen Energy Co._ Ltd. RSM72-6-315P | Risen Energy Co._ Ltd. RSM72-6-320M | Risen Energy Co._ Ltd. RSM72-6-320P | Risen Energy Co._ Ltd. RSM72-6-325M | Risen Energy Co._ Ltd. RSM72-6-325P | Risen Energy Co._ Ltd. RSM72-6-330M | Risen Energy Co._ Ltd. RSM72-6-330P | Risen Energy Co._ Ltd. RSM72-6-335M | Risen Energy Co._ Ltd. RSM72-6-335P | Risen Energy Co._ Ltd. RSM72-6-340M | Risen Energy Co._ Ltd. RSM72-6-340P | Risen Energy Co._ Ltd. RSM72-6-345M | Risen Energy Co._ Ltd. RSM72-6-345P | Risen Energy Co._ Ltd. RSM72-6-350M | Ritek PM130 | Ritek MM135 | Ritek PM135 | Ritek MM140 | Ritek PM140 | Ritek MM145 | Ritek PM175 | Ritek MM180 | Ritek PM180 | Ritek MM185 | Ritek PM185 | Ritek MM190 | Ritek PM190 | Ritek MM195 | Ritek PM195 | Ritek MM200 | Ritek PM200 | Ritek MM205 | Ritek PM205 | Ritek MM210 | Ritek PM210 | Ritek MM215 | Ritek PM215 | Ritek MM220 | Ritek PM220 | Ritek MM225 | Ritek PM225 | Ritek MM230 | Ritek PM230 | Ritek MM235 | Ritek PM235 | Ritek MM240 | Ritek PM240 | Ritek PM60-6RT-240 | Ritek PM245 | Ritek PM60-6RT-245 | Ritek MM60-6RT-250 | Ritek PM250 | Ritek PM60-6RT-250 | Ritek MM60-6RT-255 | Ritek PM255 | Ritek PM60-6RT-255 | Ritek MM60-6RT-260 | Ritek PM60-6RT-260 | Ritek MM60-6RT-265 | Ritek PM60-6RT-265 | Ritek MM60-6RT-270 | Ritek PM270T | Ritek PM60-6RT-270 | Ritek MM60-6RT-275 | Ritek PM275 | Ritek PM275T | Ritek PM60-6RT-275 | Ritek MM60-6RT-280 | Ritek PM280 | Ritek PM280T | Ritek PM60-6RT-280 | Ritek MM285T | Ritek MM60-6RT-285 | Ritek PM285 | Ritek PM285T | Ritek PM60-6RT-285 | Ritek PM72-6RT-285 | Ritek MM290T | Ritek MM60-6RT-290 | Ritek PM290 | Ritek PM290T | Ritek PM72-6RT-290 | Ritek MM295T | Ritek MM60-6RT-295 | Ritek PM295 | Ritek PM72-6RT-295 | Ritek MM300T | Ritek MM72-6RT-300 | Ritek PM72-6RT-300 | Ritek MM305T | Ritek MM72-6RT-305 | Ritek PM72-6RT-305 | Ritek MM72-6RT-310 | Ritek PM72-6RT-310 | Ritek MM72-6RT-315 | Ritek PM72-6RT-315 | Ritek MM72-6RT-320 | Ritek PM72-6RT-320 | Ritek MM72-6RT-325 | Ritek PM72-6RT-325 | Ritek MM72-6RT-330 | Ritek PM72-6RT-330 | Ritek MM72-6RT-335 | Ritek PM72-6RT-335 | Ritek MM72-6RT-340 | Ritek PM72-6RT-340 | Ritek MM72-6RT-345 | Ritek MM72-6RT-350 | Ritek MM72-6RT-355 | RSI Holding RSI-6M-250M-60 | RSI Holding RSI-6M-255M-60 | RSI Holding RSI-6M-260M-60 | RSI Holding RSI-6M-265M-60 | RSI Holding RSI-6M-270M-60 | Saga Solar S-255M60-B | Saga Solar S-260M60 | Saga Solar S-260M60-B | Saga Solar S-265M60 | Saga Solar S-265M60-B | Saga Solar S-270M60 | Saga Solar S-270M60-B | Saga Solar S-275M60 | Saga Solar S-275M60-B | Saga Solar S-280M60 | Saga Solar S-310P72 | Saga Solar S-315P72 | Saga Solar S-320P72 | Saga Solar S-325P72 | Saga Solar S-330P72 | Saint Gobain Solar SKA180M72-WN | Saint Gobain Solar SKA185M72-WN | Saint Gobain Solar SKA190M72-WN | Saint Gobain Solar SKA220P60-WN | Saint Gobain Solar SKA225M60-WN | Saint Gobain Solar SKA225P60-WN | Saint Gobain Solar SKA230M60-WN | Saint Gobain Solar SKA230P60-WN | Saint Gobain Solar SKA235P60-WN | Saint Gobain Solar SKA240M60-WN | Saint Gobain Solar SKA240P60-WN | Saint Gobain Solar SKA245M60-WN | Saint Gobain Solar SKA250M60-WN | Samsung SDI LPC235SM-02 | Samsung SDI LPC235SM-08 | Samsung SDI LPC238SM-02 | Samsung SDI LPC238SM-08 | Samsung SDI LPC241SM-02 | Samsung SDI LPC241SM-08 | Samsung SDI LPC244SM-02 | Samsung SDI LPC244SM-08 | Samsung SDI PV-MBA1BG244 | Samsung SDI PV-MBA1CG244 | Samsung SDI LPC247SM-08 | Samsung SDI PV-MBA1BG247 | Samsung SDI PV-MBA1CG247 | Samsung SDI LPC250SM-08 | Samsung SDI PV-MBA1BG250 | Samsung SDI PV-MBA1CG250 | Samsung SDI PV-MBA1BG255 | Samsung SDI PV-MBA1CG255 | SANYO ELECTRIC CO LTD OF PANASONIC GROUP HIP-186DA3 | SANYO ELECTRIC CO LTD OF PANASONIC GROUP VBHB186DA03 | SANYO ELECTRIC CO LTD OF PANASONIC GROUP VBHB186DA03B | SANYO ELECTRIC CO LTD OF PANASONIC GROUP HIP-190DA3 | SANYO ELECTRIC CO LTD OF PANASONIC GROUP VBHB190DA03 | SANYO ELECTRIC CO LTD OF PANASONIC GROUP VBHB190DA03B | SANYO ELECTRIC CO LTD OF PANASONIC GROUP HIP-195BA20 | SANYO ELECTRIC CO LTD OF PANASONIC GROUP HIP-195DA3 | SANYO ELECTRIC CO LTD OF PANASONIC GROUP VBHB195AA20 | SANYO ELECTRIC CO LTD OF PANASONIC GROUP VBHB195AA20B | SANYO ELECTRIC CO LTD OF PANASONIC GROUP VBHB195DA03 | SANYO ELECTRIC CO LTD OF PANASONIC GROUP VBHB195DA03B | SANYO ELECTRIC CO LTD OF PANASONIC GROUP HIP-200BA20 | SANYO ELECTRIC CO LTD OF PANASONIC GROUP VBHB200AA20 | SANYO ELECTRIC CO LTD OF PANASONIC GROUP VBHB200AA20B | SANYO ELECTRIC CO LTD OF PANASONIC GROUP HIT-N210A01 | SANYO ELECTRIC CO LTD OF PANASONIC GROUP VBHN210AA01 | SANYO ELECTRIC CO LTD OF PANASONIC GROUP VBHN210AA01B | SANYO ELECTRIC CO LTD OF PANASONIC GROUP HIP-215NKHA6 | SANYO ELECTRIC CO LTD OF PANASONIC GROUP HIT-N215A01 | SANYO ELECTRIC CO LTD OF PANASONIC GROUP VBHN215AA01 | SANYO ELECTRIC CO LTD OF PANASONIC GROUP VBHN215AA01B | SANYO ELECTRIC CO LTD OF PANASONIC GROUP VBHN215AA06 | SANYO ELECTRIC CO LTD OF PANASONIC GROUP VBHN215AA06B | SANYO ELECTRIC CO LTD OF PANASONIC GROUP HIT-N220A01 | SANYO ELECTRIC CO LTD OF PANASONIC GROUP VBHN220AA01 | SANYO ELECTRIC CO LTD OF PANASONIC GROUP VBHN220AA01B | SANYO ELECTRIC CO LTD OF PANASONIC GROUP VBHN220DA02 | SANYO ELECTRIC CO LTD OF PANASONIC GROUP VBHN220DA02B | SANYO ELECTRIC CO LTD OF PANASONIC GROUP VBHN220SA06 | SANYO ELECTRIC CO LTD OF PANASONIC GROUP VBHN220SA06B | SANYO ELECTRIC CO LTD OF PANASONIC GROUP HIT-N225A01 | SANYO ELECTRIC CO LTD OF PANASONIC GROUP VBHN225AA01 | SANYO ELECTRIC CO LTD OF PANASONIC GROUP VBHN225AA01B | SANYO ELECTRIC CO LTD OF PANASONIC GROUP VBHN225DA02 | SANYO ELECTRIC CO LTD OF PANASONIC GROUP VBHN225DA02B | SANYO ELECTRIC CO LTD OF PANASONIC GROUP VBHN225SA06 | SANYO ELECTRIC CO LTD OF PANASONIC GROUP VBHN225SA06B | SANYO ELECTRIC CO LTD OF PANASONIC GROUP VBHN230DA02 | SANYO ELECTRIC CO LTD OF PANASONIC GROUP VBHN230DA02B | SANYO ELECTRIC CO LTD OF PANASONIC GROUP VBHN230SA04 | SANYO ELECTRIC CO LTD OF PANASONIC GROUP VBHN230SA04B | SANYO ELECTRIC CO LTD OF PANASONIC GROUP VBHN230SA06 | SANYO ELECTRIC CO LTD OF PANASONIC GROUP VBHN230SA06B | SANYO ELECTRIC CO LTD OF PANASONIC GROUP VBHN230SA11 | SANYO ELECTRIC CO LTD OF PANASONIC GROUP VBHN230SA11B | SANYO ELECTRIC CO LTD OF PANASONIC GROUP VBHN235SA04 | SANYO ELECTRIC CO LTD OF PANASONIC GROUP VBHN235SA04B | SANYO ELECTRIC CO LTD OF PANASONIC GROUP VBHN235SA06 | SANYO ELECTRIC CO LTD OF PANASONIC GROUP VBHN235SA06B | SANYO ELECTRIC CO LTD OF PANASONIC GROUP VBHN235SA11 | SANYO ELECTRIC CO LTD OF PANASONIC GROUP VBHN235SA11B | SANYO ELECTRIC CO LTD OF PANASONIC GROUP VBHN240SA04 | SANYO ELECTRIC CO LTD OF PANASONIC GROUP VBHN240SA04B | SANYO ELECTRIC CO LTD OF PANASONIC GROUP VBHN240SA06 | SANYO ELECTRIC CO LTD OF PANASONIC GROUP VBHN240SA06B | SANYO ELECTRIC CO LTD OF PANASONIC GROUP VBHN240SA11 | SANYO ELECTRIC CO LTD OF PANASONIC GROUP VBHN240SA11B | SANYO ELECTRIC CO LTD OF PANASONIC GROUP VBMS240AA02 | SANYO ELECTRIC CO LTD OF PANASONIC GROUP VBHN245SA04 | SANYO ELECTRIC CO LTD OF PANASONIC GROUP VBHN245SA04B | SANYO ELECTRIC CO LTD OF PANASONIC GROUP VBHN245SA06 | SANYO ELECTRIC CO LTD OF PANASONIC GROUP VBHN245SA06B | SANYO ELECTRIC CO LTD OF PANASONIC GROUP VBHN245SA11 | SANYO ELECTRIC CO LTD OF PANASONIC GROUP VBHN245SA11B | SANYO ELECTRIC CO LTD OF PANASONIC GROUP VBMS245AA02 | SANYO ELECTRIC CO LTD OF PANASONIC GROUP VBMS250AA02 | SANYO ELECTRIC CO LTD OF PANASONIC GROUP VBMS250AA04 | SANYO ELECTRIC CO LTD OF PANASONIC GROUP VBMS255AA04 | SANYO ELECTRIC CO LTD OF PANASONIC GROUP VBMS260AA04 | SANYO ELECTRIC CO LTD OF PANASONIC GROUP VBHN307ZA04 | SANYO ELECTRIC CO LTD OF PANASONIC GROUP VBHN310KA01 | SANYO ELECTRIC CO LTD OF PANASONIC GROUP VBHN310KA03 | SANYO ELECTRIC CO LTD OF PANASONIC GROUP VBHN310ZA03 | SANYO ELECTRIC CO LTD OF PANASONIC GROUP VBHN310ZA04 | SANYO ELECTRIC CO LTD OF PANASONIC GROUP VBHN315KA01 | SANYO ELECTRIC CO LTD OF PANASONIC GROUP VBHN315KA03 | SANYO ELECTRIC CO LTD OF PANASONIC GROUP VBHN315ZA03 | SANYO ELECTRIC CO LTD OF PANASONIC GROUP VBHN315ZA04 | SANYO ELECTRIC CO LTD OF PANASONIC GROUP VBHN320KA01 | SANYO ELECTRIC CO LTD OF PANASONIC GROUP VBHN320KA03 | SANYO ELECTRIC CO LTD OF PANASONIC GROUP VBHN320SA15 | SANYO ELECTRIC CO LTD OF PANASONIC GROUP VBHN320SA15B | SANYO ELECTRIC CO LTD OF PANASONIC GROUP VBHN320SA16 | SANYO ELECTRIC CO LTD OF PANASONIC GROUP VBHN320SA16B | SANYO ELECTRIC CO LTD OF PANASONIC GROUP VBHN320ZA01 | SANYO ELECTRIC CO LTD OF PANASONIC GROUP VBHN320ZA03 | SANYO ELECTRIC CO LTD OF PANASONIC GROUP VBHN325KA03 | SANYO ELECTRIC CO LTD OF PANASONIC GROUP VBHN325SA15 | SANYO ELECTRIC CO LTD OF PANASONIC GROUP VBHN325SA15B | SANYO ELECTRIC CO LTD OF PANASONIC GROUP VBHN325SA16 | SANYO ELECTRIC CO LTD OF PANASONIC GROUP VBHN325SA16B | SANYO ELECTRIC CO LTD OF PANASONIC GROUP VBHN325SA17 | SANYO ELECTRIC CO LTD OF PANASONIC GROUP VBHN325ZA01 | SANYO ELECTRIC CO LTD OF PANASONIC GROUP VBHN330SA15 | SANYO ELECTRIC CO LTD OF PANASONIC GROUP VBHN330SA15B | SANYO ELECTRIC CO LTD OF PANASONIC GROUP VBHN330SA16 | SANYO ELECTRIC CO LTD OF PANASONIC GROUP VBHN330SA16B | SANYO ELECTRIC CO LTD OF PANASONIC GROUP VBHN330SA17 | SANYO ELECTRIC CO LTD OF PANASONIC GROUP VBHN330ZA01 | SANYO ELECTRIC CO LTD OF PANASONIC GROUP VBHN332SA16 | SANYO ELECTRIC CO LTD OF PANASONIC GROUP VBHN332SA16B | SANYO ELECTRIC CO LTD OF PANASONIC GROUP VBHN333SA16 | SANYO ELECTRIC CO LTD OF PANASONIC GROUP VBHN333SA16B | SANYO ELECTRIC CO LTD OF PANASONIC GROUP VBHN335SA16 | SANYO ELECTRIC CO LTD OF PANASONIC GROUP VBHN335SA16B | SANYO ELECTRIC CO LTD OF PANASONIC GROUP VBHN335SA17 | Scheuten Solar Logistics P6-60i30-200 | Scheuten Solar Logistics P6-60i30-205 | Scheuten Solar Logistics P6-60i30-210 | Scheuten Solar Logistics P6-60i30-215 | Scheuten Solar Logistics P6-60i30-220 | Scheuten Solar Logistics P6-60i30-225 | Scheuten Solar Logistics P6-60i30-230 | Scheuten Solar Logistics P6-60i30-235 | Scheuten Solar Logistics P6-60i30-240 | Scheuten Solar USA P6-54 185W | Scheuten Solar USA P6-54 190W | Scheuten Solar USA P6-54 195W | Scheuten Solar USA P6-54 200W | Scheuten Solar USA P6-54 205W | Scheuten Solar USA P6-60U-210W | Scheuten Solar USA P6-60U-215W | Scheuten Solar USA P6-60U-220W | Scheuten Solar USA P6-60U-225W | Scheuten Solar USA P6-60U-230W | Scheuten Solar USA P6-60U-235W | Scheuten Solar USA P6-60U-240W | Schott Solar ASE-300-DGF/25-145 | Schott Solar SAPC-165 | Schott Solar SAPC-165S | Schott Solar SAPC-170 | Schott Solar SAPC-175 | Schott Solar ASE-300-DGF/34-195 | Schott Solar Perform Poly 202 | Schott Solar Poly 202 | Schott Solar Perform Poly 210 | Schott Solar Poly 210 | Schott Solar Perform Poly 217 | Schott Solar Poly 217 | Schott Solar Perform Poly 220 | Schott Solar Poly 220 | Schott Solar Perform Poly 225 | Schott Solar Poly 225 | Schott Solar Perform Poly 230 | Schott Solar Poly 230 | Schott Solar Perform Poly 235 | Schott Solar Poly 235 | Schott Solar ASE-300-DGF/42-240 | Schott Solar Perform Mono 240 | Schott Solar Perform Poly 240 | Schott Solar Poly 240 | Schott Solar Perform Mono 245 | Schott Solar PERFORM POLY 245 | Schott Solar ASE-300-DGF/50-250 | Schott Solar Perform Mono 250 | Schott Solar PERFORM POLY 250 | Schott Solar Perform Mono 255 | Schott Solar ASE-300-DGF/50-260 | Schott Solar Perform Mono 260 | Schott Solar ASE-300-DGF/50-270 | Schott Solar ASE-300-DGF/50-280 | Schott Solar ASE-300-DGF/50-290 | Schott Solar ASE-300-DGF/50-300 | Schott Solar ASE-300-DGF/50-310 | Schuco International MPE 235 PS03 | Schuco International MPE 310 MP 02 | Schuco International MPE 320 MP 02 | Schuco USA MPE 85 AL 01 | Schuco USA MPE 90 AL 01 | Schuco USA S 165-SPU | Schuco USA S 165-SPU-4 | Schuco USA MPE 170 MS 05 | Schuco USA S 170-SPU | Schuco USA S 170-SPU-4 | Schuco USA MPE 175 MS 05 | Schuco USA S 175-SPU-4 | Schuco USA MPE 180 MS 05 | Schuco USA S 180-SPU-4 | Schuco USA MPE 185 MS 05 | Schuco USA MPE 190 MS 05 | Schuco USA MPE 200 PS 04 | Schuco USA MPE 205 PS 04 | Schuco USA MPE 210 PS 04 | Schuco USA MPE 215 PS 04 | Schuco USA MPE 220 PS 04 | Schuco USA MPE 220 PS 09 | Schuco USA MPE 225 PS 04 | Schuco USA MPE 225 PS 08 | Schuco USA MPE 225 PS 09 | Schuco USA MPE 225 PS 60 BA | Schuco USA MPE 230 PS 04 | Schuco USA MPE 230 PS 08 | Schuco USA MPE 230 PS 09 | Schuco USA MPE 230 PS 60 BA | Schuco USA MPE 235 PS 08 | Schuco USA MPE 235 PS 09 | Schuco USA MPE 235 PS 60 BA | Schuco USA MPE 240 MS 08 | Schuco USA MPE 240 MS 60 BA | Schuco USA MPE 240 MS 60 BB | Schuco USA MPE 240 PS 08 | Schuco USA MPE 240 PS 09 | Schuco USA MPE 255 PS 60 BA | Schuco USA MPE 245 MS 08 | Schuco USA MPE 245 MS 60 BA | Schuco USA MPE 245 MS 60 BB | Schuco USA MPE 245 PS 08 | Schuco USA MPE 245 PS 60 BA | Schuco USA MPE 250 MS 08 | Schuco USA MPE 250 MS 60 BA | Schuco USA MPE 250 MS 60 BB | Schuco USA MPE 250 PS 60 BA | Schuco USA MPE 240 PS 60 BA | Schuco USA MPE 255 MS 08 | Schuco USA MPE 255 MS 60 BA | Schuco USA MPE 255 MS 60 BB | Schuco USA MPE 260 MS 08 | Schuco USA MPE 260 MS 60 BA | Schuco USA MPE 260 MS 60 BB | Schuco USA MPE 260 PS 60 BA | Schuco USA MPE 265 MS 08 | Schuco USA MPE 265 MS 60 BA | Schuco USA MPE 265 MS 60 BB | Schuco USA MPE 270 MS 08 | Schuco USA MPE 270 MS 60 BA | Schuco USA MPE 270 MS 60 BB | Schuco USA MPE 350 AL 01 | Schuco USA MPE 360 AL 01 | Semyung Electric SM-T-390-Platinum | Semyung Electric SM-T-395-Platinum | Semyung Electric SM-T-400-Platinum | Semyung Electric SM-T-405-Platinum | Semyung Electric SM-T-410-Platinum | S-Energy Co._ Ltd. SM-200MC1 | S-Energy Co._ Ltd. SM-205MC1 | S-Energy Co._ Ltd. SM-210MC1 | S-Energy Co._ Ltd. SM-215MC1 | S-Energy Co._ Ltd. SM-215PC5 | S-Energy Co._ Ltd. SM-220MC1 | S-Energy Co._ Ltd. SM-220PC5 | S-Energy Co._ Ltd. SM-225MC1 | S-Energy Co._ Ltd. SM-225PC5 | S-Energy Co._ Ltd. SM-230MC1 | S-Energy Co._ Ltd. SM-230PC5 | S-Energy Co._ Ltd. SM-230PC8 | S-Energy Co._ Ltd. SM-235MC1 | S-Energy Co._ Ltd. SM-235PC5 | S-Energy Co._ Ltd. SM-235PC8 | S-Energy Co._ Ltd. SM-240PC8 | S-Energy Co._ Ltd. SM-245PC8 | S-Energy Co._ Ltd. SN245P-10 | S-Energy Co._ Ltd. SN245P-15 | S-Energy Co._ Ltd. SM-250PC8 | S-Energy Co._ Ltd. SN250P-10 | S-Energy Co._ Ltd. SN250P-15 | S-Energy Co._ Ltd. SM-255PC8 | S-Energy Co._ Ltd. SN255P-10 | S-Energy Co._ Ltd. SN255P-15 | S-Energy Co._ Ltd. SM-260PC8 | S-Energy Co._ Ltd. SN260P-10 | S-Energy Co._ Ltd. SN260P-15 | S-Energy Co._ Ltd. SM-265PC5 | S-Energy Co._ Ltd. SN265P-10 | S-Energy Co._ Ltd. SN265P-15 | S-Energy Co._ Ltd. SM-270PC5 | S-Energy Co._ Ltd. SN270P-10 | S-Energy Co._ Ltd. SM-275PC5 | S-Energy Co._ Ltd. SM-275PC8 | S-Energy Co._ Ltd. SN275M-10(B) | S-Energy Co._ Ltd. SM-280PC5 | S-Energy Co._ Ltd. SM-280PC8 | S-Energy Co._ Ltd. SN280M-10 | S-Energy Co._ Ltd. SN280M-10(B) | S-Energy Co._ Ltd. SM-285PC5 | S-Energy Co._ Ltd. SM-285PC8 | S-Energy Co._ Ltd. SN285M-10 | S-Energy Co._ Ltd. SN285M-10(B) | S-Energy Co._ Ltd. SM-290PC8 | S-Energy Co._ Ltd. SN290M-10 | S-Energy Co._ Ltd. SN290M-10(B) | S-Energy Co._ Ltd. SM-295PC8 | S-Energy Co._ Ltd. SN295M-10 | S-Energy Co._ Ltd. SN295M-10(B) | S-Energy Co._ Ltd. SN295P-10 | S-Energy Co._ Ltd. SN295P-15 | S-Energy Co._ Ltd. SM-300PC8 | S-Energy Co._ Ltd. SN300M-10 | S-Energy Co._ Ltd. SN300M-10(B) | S-Energy Co._ Ltd. SN300P-10 | S-Energy Co._ Ltd. SN300P-15 | S-Energy Co._ Ltd. SM-305PC8 | S-Energy Co._ Ltd. SN305M-10(B) | S-Energy Co._ Ltd. SN305P-10 | S-Energy Co._ Ltd. SN305P-15 | S-Energy Co._ Ltd. SN310M-10(B) | S-Energy Co._ Ltd. SN310P-10 | S-Energy Co._ Ltd. SN310P-15 | S-Energy Co._ Ltd. SN315P-10 | S-Energy Co._ Ltd. SN315P-15 | S-Energy Co._ Ltd. SN320P-10 | S-Energy Co._ Ltd. SN320P-15 | S-Energy Co._ Ltd. SN325P-10 | S-Energy Co._ Ltd. SN325P-15 | S-Energy Co._ Ltd. SN330M-10(B) | S-Energy Co._ Ltd. SN335M-10(B) | S-Energy Co._ Ltd. SN340M-10 | S-Energy Co._ Ltd. SN340M-10(B) | S-Energy Co._ Ltd. SN345M-10 | S-Energy Co._ Ltd. SN345M-10(B) | S-Energy Co._ Ltd. SN350M-10 | S-Energy Co._ Ltd. SN350M-10(B) | S-Energy Co._ Ltd. SN355M-10 | S-Energy Co._ Ltd. SN355M-10(B) | S-Energy Co._ Ltd. SN360M-10 | S-Energy Co._ Ltd. SN360M-10(B) | S-Energy Co._ Ltd. SN365M-10(B) | S-Energy Co._ Ltd. SN370M-10(B) | Seraphim Energy Group Inc. SEG-BPB-255BB | Seraphim Energy Group Inc. SEG-BPB-260BB | Seraphim Energy Group Inc. SEG-BPB-260WB | Seraphim Energy Group Inc. SEG-BPB-260WW | Seraphim Energy Group Inc. SEG-6PB-265WB | Seraphim Energy Group Inc. SEG-6PB-265WW | Seraphim Energy Group Inc. SEG-BPB-265BB | Seraphim Energy Group Inc. SEG-BPB-265WB | Seraphim Energy Group Inc. SEG-BPB-265WW | Seraphim Energy Group Inc. SEG-BPB-270BB | Seraphim Energy Group Inc. SEG-BPB-270WB | Seraphim Energy Group Inc. SEG-BPB-270WW | Seraphim Energy Group Inc. SEG-BPB-275BB | Seraphim Energy Group Inc. SEG-BPB-275WB | Seraphim Energy Group Inc. SEG-BPB-275WW | Seraphim Energy Group Inc. SEG-6MB-280BB | Seraphim Energy Group Inc. SEG-BMB-280BB | Seraphim Energy Group Inc. SEG-BPB-280BB | Seraphim Energy Group Inc. SEG-BPB-280WB | Seraphim Energy Group Inc. SEG-BPB-280WW | Seraphim Energy Group Inc. SEG-6MB-285BB | Seraphim Energy Group Inc. SEG-BMB-285BB | Seraphim Energy Group Inc. SEG-BPB-285WB | Seraphim Energy Group Inc. SEG-BPB-285WW | Seraphim Energy Group Inc. SEG-E11B-285 | Seraphim Energy Group Inc. SEG-6MB-290BB | Seraphim Energy Group Inc. SEG-BMB-290BB | Seraphim Energy Group Inc. SEG-BMB-290WB | Seraphim Energy Group Inc. SEG-BMB-290WW | Seraphim Energy Group Inc. SEG-E11B-290 | Seraphim Energy Group Inc. SEG-6MB-295BB | Seraphim Energy Group Inc. SEG-BMB-295BB | Seraphim Energy Group Inc. SEG-BMB-295WB | Seraphim Energy Group Inc. SEG-BMB-295WW | Seraphim Energy Group Inc. SEG-E11B-295 | Seraphim Energy Group Inc. SEG-BMB-300BB | Seraphim Energy Group Inc. SEG-BMB-300WB | Seraphim Energy Group Inc. SEG-BMB-300WW | Seraphim Energy Group Inc. SEG-E01B-300 | Seraphim Energy Group Inc. SEG-E11B-300 | Seraphim Energy Group Inc. SEG-BMB-305BB | Seraphim Energy Group Inc. SEG-BMB-305WB | Seraphim Energy Group Inc. SEG-BMB-305WW | Seraphim Energy Group Inc. SEG-E01B-305 | Seraphim Energy Group Inc. SEG-E11B-305 | Seraphim Energy Group Inc. SEG-BMB-310BB | Seraphim Energy Group Inc. SEG-BMB-310WB | Seraphim Energy Group Inc. SEG-BMB-310WW | Seraphim Energy Group Inc. SEG-BPA-310WW | Seraphim Energy Group Inc. SEG-E01B-310 | Seraphim Energy Group Inc. SEG-E11B-310 | Seraphim Energy Group Inc. SEG-BPA-315WW | Seraphim Energy Group Inc. SEG-E01B-315 | Seraphim Energy Group Inc. SEG-6PA-320WW | Seraphim Energy Group Inc. SEG-BPA-320WW | Seraphim Energy Group Inc. SEG-BPA-325WW | Seraphim Energy Group Inc. SEG-E01B-325 | Seraphim Energy Group Inc. SEG-BPA-330WW | Seraphim Energy Group Inc. SEG-E01B-330 | Seraphim Energy Group Inc. SEG-6MA-335WW | Seraphim Energy Group Inc. SEG-BPA-335WW | Seraphim Energy Group Inc. SEG-6MA-340WW | Seraphim Energy Group Inc. SEG-BMA-340WW | Seraphim Energy Group Inc. SEG-BPA-340WW | Seraphim Energy Group Inc. SEG-6MA-345WW | Seraphim Energy Group Inc. SEG-BMA-345WW | Seraphim Energy Group Inc. SEG-BPA-345WW | Seraphim Energy Group Inc. SEG-E11A-345 | Seraphim Energy Group Inc. SEG-6MA-350WW | Seraphim Energy Group Inc. SEG-BMA-350WW | Seraphim Energy Group Inc. SEG-6MA-355WW | Seraphim Energy Group Inc. SEG-BMA-355WW | Seraphim Energy Group Inc. SEG-6MA-360WW | Seraphim Energy Group Inc. SEG-BMA-360WW | Seraphim Energy Group Inc. SEG-E11A-360 | Seraphim Energy Group Inc. SEG-BMA-365WW | Seraphim Energy Group Inc. SEG-E01A-365 | Seraphim Energy Group Inc. SEG-BMA-370WW | Seraphim Energy Group Inc. SEG-E11A-370 | Seraphim Energy Group Inc. SEG-BMA-375WW | Seraphim Energy Group Inc. SEG-E11A-375 | Seraphim Energy Group Inc. SEG-E01A-385 | Seraphim Energy Group Inc. SEG-E01A-390 | Seraphim Solar System Co._Ltd. SRP-180-5MB | Seraphim Solar System Co._Ltd. SRP-185-5MB | Seraphim Solar System Co._Ltd. SRP-190-5MB | Seraphim Solar System Co._Ltd. SRP-195-5MB | Seraphim Solar System Co._Ltd. SRP-200-5MB | Seraphim Solar System Co._Ltd. SRP-205-5MB | Seraphim Solar System Co._Ltd. SRP-210-5MB | Seraphim Solar System Co._Ltd. SRP-220-6PC | Seraphim Solar System Co._Ltd. SRP-225-6PC | Seraphim Solar System Co._Ltd. SRP-230-6PB | Seraphim Solar System Co._Ltd. SRP-230-6PC | Seraphim Solar System Co._Ltd. SRP-235-6MC | Seraphim Solar System Co._Ltd. SRP-235-6PB | Seraphim Solar System Co._Ltd. SRP-235-6PC | Seraphim Solar System Co._Ltd. SRP-240-6MC | Seraphim Solar System Co._Ltd. SRP-240-6PB | Seraphim Solar System Co._Ltd. SRP-240-6PC | Seraphim Solar System Co._Ltd. SRP-245-6MC | Seraphim Solar System Co._Ltd. SRP-245-6PB | Seraphim Solar System Co._Ltd. SRP-250-6MC | Seraphim Solar System Co._Ltd. SRP-250-6PB | Seraphim Solar System Co._Ltd. SRP-255-6MC | Seraphim Solar System Co._Ltd. SRP-255-6PB | Seraphim Solar System Co._Ltd. SRP-260-6MB | Seraphim Solar System Co._Ltd. SRP-260-6PB | Seraphim Solar System Co._Ltd. SRP-265-5MA | Seraphim Solar System Co._Ltd. SRP-265-6MB | Seraphim Solar System Co._Ltd. SRP-265-6PB | Seraphim Solar System Co._Ltd. SRP-270-5MA | Seraphim Solar System Co._Ltd. SRP-270-6MB | Seraphim Solar System Co._Ltd. SRP-270-6PB | Seraphim Solar System Co._Ltd. SRP-275-5MA | Seraphim Solar System Co._Ltd. SRP-275-6MB | Seraphim Solar System Co._Ltd. SRP-275-6PA | Seraphim Solar System Co._Ltd. SRP-275-6PB | Seraphim Solar System Co._Ltd. SRP-280-5MA | Seraphim Solar System Co._Ltd. SRP-280-6MB | Seraphim Solar System Co._Ltd. SRP-280-6PA | Seraphim Solar System Co._Ltd. SRP-285-5MA | Seraphim Solar System Co._Ltd. SRP-285-6MB | Seraphim Solar System Co._Ltd. SRP-285-6MB-BB | Seraphim Solar System Co._Ltd. SRP-285-6PA | Seraphim Solar System Co._Ltd. SRP-290-6MA | Seraphim Solar System Co._Ltd. SRP-290-6MB | Seraphim Solar System Co._Ltd. SRP-290-6MB-BB | Seraphim Solar System Co._Ltd. SRP-290-6PA | Seraphim Solar System Co._Ltd. SRP-295-6MA | Seraphim Solar System Co._Ltd. SRP-295-6MB | Seraphim Solar System Co._Ltd. SRP-295-6MB-BB | Seraphim Solar System Co._Ltd. SRP-295-6PA | Seraphim Solar System Co._Ltd. SRP-300-6MA | Seraphim Solar System Co._Ltd. SRP-300-6MB | Seraphim Solar System Co._Ltd. SRP-300-6MB-BB | Seraphim Solar System Co._Ltd. SRP-300-6PA | Seraphim Solar System Co._Ltd. SRP-305-6MA | Seraphim Solar System Co._Ltd. SRP-305-6MB-BB | Seraphim Solar System Co._Ltd. SRP-305-6PA | Seraphim Solar System Co._Ltd. SRP-310-6MA | Seraphim Solar System Co._Ltd. SRP-310-6PA | Seraphim Solar System Co._Ltd. SRP-315-6MA | Seraphim Solar System Co._Ltd. SRP-315-6PA | Seraphim Solar System Co._Ltd. SRP-320-6MA | Seraphim Solar System Co._Ltd. SRP-320-6PA | Seraphim Solar System Co._Ltd. SRP-325-6MA | Seraphim Solar System Co._Ltd. SRP-325-6PA | Seraphim Solar System Co._Ltd. SRP-330-6MA | Seraphim Solar System Co._Ltd. SRP-330-6PA | Seraphim Solar System Co._Ltd. SRP-335-6MA | Seraphim Solar System Co._Ltd. SRP-340-6MA | Seraphim Solar System Co._Ltd. SRP-345-6MA | Seraphim Solar System Co._Ltd. SRP-350-6MA | Seraphim Solar System Co._Ltd. SRP-355-6MA | Seraphim Solar System Co._Ltd. SRP-360-6MA | Seraphim Solar USA Manufacturing Inc. SRP-345-6QA-WB-40 | Seraphim Solar USA Manufacturing Inc. SRP-345-6QA-WB-50 | Seraphim Solar USA Manufacturing Inc. SRP-345-6QA-WS-40 | Seraphim Solar USA Manufacturing Inc. SRP-345-6QA-WS-50 | Seraphim Solar USA Manufacturing Inc. SRP-350-6QA-WB-40 | Seraphim Solar USA Manufacturing Inc. SRP-350-6QA-WB-50 | Seraphim Solar USA Manufacturing Inc. SRP-350-6QA-WS-40 | Seraphim Solar USA Manufacturing Inc. SRP-350-6QA-WS-50 | Seraphim Solar USA Manufacturing Inc. SRP-355-6QA-WB-40 | Seraphim Solar USA Manufacturing Inc. SRP-355-6QA-WB-50 | Seraphim Solar USA Manufacturing Inc. SRP-355-6QA-WS-40 | Seraphim Solar USA Manufacturing Inc. SRP-355-6QA-WS-50 | Seraphim Solar USA Manufacturing Inc. SRP-360-6QA-WB-40 | Seraphim Solar USA Manufacturing Inc. SRP-360-6QA-WB-50 | Seraphim Solar USA Manufacturing Inc. SRP-360-6QA-WS-40 | Seraphim Solar USA Manufacturing Inc. SRP-360-6QA-WS-50 | Seraphim Solar USA Manufacturing Inc. SRP-365-6QA-WB-40 | Seraphim Solar USA Manufacturing Inc. SRP-365-6QA-WB-50 | Seraphim Solar USA Manufacturing Inc. SRP-365-6QA-WS-40 | Seraphim Solar USA Manufacturing Inc. SRP-365-6QA-WS-50 | SET-Solar SETA-125-150W-72M | SET-Solar SETA-125-155W-72M | SET-Solar SETA-125-160W-72M | SET-Solar SDM-170/(165)-72M | SET-Solar SETA-125-165W-72M | SET-Solar SDM-170/(170)-72M | SET-Solar SETA-125-170W-72M | SET-Solar SDM-170/(175)-72M | SET-Solar SETA-125-175W-72M | SET-Solar SETB-125-175W-72M | SET-Solar SDM-170/(180)-72M | SET-Solar SETA-125-180W-72M | SET-Solar SETB-125-180W-72M | SET-Solar SETD-125-180W-72M | SET-Solar SDM-170/(185)-72M | SET-Solar SETA-125-185W-72M | SET-Solar SETB-125-185W-72M | SET-Solar SETD-125-185W-72M | SET-Solar SETB-156-190W-54P | SET-Solar SETB-156-195W-54P | SET-Solar SETB-156-200W-54P | SET-Solar SETB-156-205W-54P | SET-Solar SETB-156-210W-54P | Shandong Dahai Group DHP72-290 | Shandong Dahai Group DHP72-295 | Shandong Dahai Group DHP72-300 | Shandong Dahai Group DHP72-305 | Shandong Dahai Group DHP72-310 | Shandong Linuo Photovoltaic Hi-Tech LN180(36)M-185 | Shandong Linuo Photovoltaic Hi-Tech LN180(36)M-190 | Shandong Linuo Photovoltaic Hi-Tech LN240(30)P-220 | Shandong Linuo Photovoltaic Hi-Tech LN240(30)P-225 | Shandong Linuo Photovoltaic Hi-Tech LN240(30)P-230 | Shandong Linuo Photovoltaic Hi-Tech LN240(30)P-235 | Shandong Linuo Photovoltaic Hi-Tech LN240(30)P-240 | Shanghai Aerospace Automobile Electromechanical HT60-156P-230 | Shanghai Aerospace Automobile Electromechanical HT60-156P-235 | Shanghai Aerospace Automobile Electromechanical HT60-156P-240 | Shanghai Aerospace Automobile Electromechanical HT60-156P-245 | Shanghai Aerospace Automobile Electromechanical HT60-156P-250 | Shanghai Aerospace Automobile Electromechanical HT60-156P-255 | Shanghai Aerospace Automobile Electromechanical HT60-156P-260 | Shanghai Aerospace Automobile Electromechanical HT60-156P-265 | Shanghai Aerospace Automobile Electromechanical HT60-156P-270 | Shanghai Aerospace Automobile Electromechanical HT60-156P-275 | Shanghai Aerospace Automobile Electromechanical HT72-156P-275 | Shanghai Aerospace Automobile Electromechanical HT72-156P-280 | Shanghai Aerospace Automobile Electromechanical HT72-156P-285 | Shanghai Aerospace Automobile Electromechanical HT72-156P-290 | Shanghai Aerospace Automobile Electromechanical HT72-156P-295 | Shanghai Aerospace Automobile Electromechanical HT72-156P-300 | Shanghai Aerospace Automobile Electromechanical HT72-156P-305 | Shanghai Aerospace Automobile Electromechanical HT72-156P-310 | Shanghai Aerospace Automobile Electromechanical HT72-156P-315 | Shanghai Aerospace Automobile Electromechanical HT72-156P-320 | Shanghai Aerospace Automobile Electromechanical HT72-156P-325 | Shanghai Aerospace Automobile Electromechanical Co._ Ltd. HT60-156P(V)-260 | Shanghai Aerospace Automobile Electromechanical Co._ Ltd. HT60-156P(V)-265 | Shanghai Aerospace Automobile Electromechanical Co._ Ltd. HT60-156P(V)-270 | Shanghai Aerospace Automobile Electromechanical Co._ Ltd. HT60-156P(V)-275 | Shanghai Aerospace Automobile Electromechanical Co._ Ltd. HT60-156M(V)-280 | Shanghai Aerospace Automobile Electromechanical Co._ Ltd. HT60-156P(V)-280 | Shanghai Aerospace Automobile Electromechanical Co._ Ltd. HT60-156M(V)-285 | Shanghai Aerospace Automobile Electromechanical Co._ Ltd. HT60-156M(V)-290 | Shanghai Aerospace Automobile Electromechanical Co._ Ltd. HT60-156M(V)-295 | Shanghai Aerospace Automobile Electromechanical Co._ Ltd. HT60-156M(V)-300 | Shanghai Aerospace Automobile Electromechanical Co._ Ltd. HT72-156P(V)-310 | Shanghai Aerospace Automobile Electromechanical Co._ Ltd. HT72-156P(V)-315 | Shanghai Aerospace Automobile Electromechanical Co._ Ltd. HT72-156P(V)-320 | Shanghai Aerospace Automobile Electromechanical Co._ Ltd. HT72-156P(V)-325 | Shanghai Aerospace Automobile Electromechanical Co._ Ltd. HT72-156P(V)-330 | Shanghai Aerospace Automobile Electromechanical Co._ Ltd. HT72-156P(V)-335 | Shanghai Aerospace Automobile Electromechanical Co._ Ltd. HT72-156M(V)-340 | Shanghai Aerospace Automobile Electromechanical Co._ Ltd. HT72-156P(V)-340 | Shanghai Aerospace Automobile Electromechanical Co._ Ltd. HT72-156M(V)-345 | Shanghai Aerospace Automobile Electromechanical Co._ Ltd. HT72-156M(V)-350 | Shanghai Aerospace Automobile Electromechanical Co._ Ltd. HT72-156M(V)-355 | Shanghai Aerospace Automobile Electromechanical Co._ Ltd. HT72-156M(V)-360 | Shanghai Aerospace Automobile Electromechanical Co._ Ltd. HT72-156M(V)-365 | Shanghai Aerospace Automobile Electromechanical Co._ Ltd. HT72-156M(V)-370 | Shanghai Alex Solar Energy Science & Technology ALM-170D-24 | Shanghai Alex Solar Energy Science & Technology ALM-175D-24 | Shanghai Alex Solar Energy Science & Technology ALM-180D-24 | Shanghai Chaori Solar Energy Science & Technology CRM60S125M-24 | Shanghai Chaori Solar Energy Science & Technology CRM60S125S | Shanghai Chaori Solar Energy Science & Technology CRM85S125M-36 | Shanghai Chaori Solar Energy Science & Technology CRM85S125S | Shanghai Chaori Solar Energy Science & Technology CRM115S125M-48 | Shanghai Chaori Solar Energy Science & Technology CRM115S125S | Shanghai Chaori Solar Energy Science & Technology CRM145S125M-60 | Shanghai Chaori Solar Energy Science & Technology CRM145S125S | Shanghai Chaori Solar Energy Science & Technology CRM175S125M-72 | Shanghai Chaori Solar Energy Science & Technology CRM175S125S | Shanghai Chaori Solar Energy Science & Technology CRM180S125M-72 | Shanghai Chaori Solar Energy Science & Technology CRM185S125M-72 | Shanghai Chaori Solar Energy Science & Technology CRM185S156P-54(T) | Shanghai Chaori Solar Energy Science & Technology CRM190S125M-72 | Shanghai Chaori Solar Energy Science & Technology CRM190S156P-54(T) | Shanghai Chaori Solar Energy Science & Technology CRM195S125M-72 | Shanghai Chaori Solar Energy Science & Technology CRM195S125M-80 | Shanghai Chaori Solar Energy Science & Technology CRM195S125S | Shanghai Chaori Solar Energy Science & Technology CRM195S156P-54(T) | Shanghai Chaori Solar Energy Science & Technology CRM200S156P-54(T) | Shanghai Chaori Solar Energy Science & Technology CRM200S156P-60(T) | Shanghai Chaori Solar Energy Science & Technology CRM205S125M-80 | Shanghai Chaori Solar Energy Science & Technology CRM205S156P-54(T) | Shanghai Chaori Solar Energy Science & Technology CRM205S156P-60(T) | Shanghai Chaori Solar Energy Science & Technology CRM210S125M-80 | Shanghai Chaori Solar Energy Science & Technology CRM210S156P-54(T) | Shanghai Chaori Solar Energy Science & Technology CRM210S156P-60(T) | Shanghai Chaori Solar Energy Science & Technology CRM215S125M-80 | Shanghai Chaori Solar Energy Science & Technology CRM215S156P-54(T) | Shanghai Chaori Solar Energy Science & Technology CRM215S156P-60(T) | Shanghai Chaori Solar Energy Science & Technology CRM220S156P-54(T) | Shanghai Chaori Solar Energy Science & Technology CRM220S156P-60(T) | Shanghai Chaori Solar Energy Science & Technology CRM225S156P-54(T) | Shanghai Chaori Solar Energy Science & Technology CRM225S156P-60(T) | Shanghai Chaori Solar Energy Science & Technology CRM230S156P-54(T) | Shanghai Chaori Solar Energy Science & Technology CRM230S156P-60(T) | Shanghai Chaori Solar Energy Science & Technology CRM235S125M-96 | Shanghai Chaori Solar Energy Science & Technology CRM235S125S | Shanghai Chaori Solar Energy Science & Technology CRM235S156P-60(T) | Shanghai Chaori Solar Energy Science & Technology CRM240S125M-96 | Shanghai Chaori Solar Energy Science & Technology CRM240S156P-60(T) | Shanghai Chaori Solar Energy Science & Technology CRM240S156P-72(T) | Shanghai Chaori Solar Energy Science & Technology CRM245S125M-96 | Shanghai Chaori Solar Energy Science & Technology CRM245S156P-60(T) | Shanghai Chaori Solar Energy Science & Technology CRM245S156P-72(T) | Shanghai Chaori Solar Energy Science & Technology CRM250S125M-96 | Shanghai Chaori Solar Energy Science & Technology CRM250S156P-60(T) | Shanghai Chaori Solar Energy Science & Technology CRM250S156P-72(T) | Shanghai Chaori Solar Energy Science & Technology CRM255S125M-96 | Shanghai Chaori Solar Energy Science & Technology CRM255S156P-60(T) | Shanghai Chaori Solar Energy Science & Technology CRM255S156P-72(T) | Shanghai Chaori Solar Energy Science & Technology CRM260S125M-96 | Shanghai Chaori Solar Energy Science & Technology CRM260S156P-60(T) | Shanghai Chaori Solar Energy Science & Technology CRM260S156P-72(T) | Shanghai Chaori Solar Energy Science & Technology CRM265S125M-96 | Shanghai Chaori Solar Energy Science & Technology CRM265S156P-72(T) | Shanghai Chaori Solar Energy Science & Technology CRM270S156P-72(T) | Shanghai Chaori Solar Energy Science & Technology CRM275S156P-72(T) | Shanghai Chaori Solar Energy Science & Technology CRM280S156P-72(T) | Shanghai Chaori Solar Energy Science & Technology CRM285S156P-72(T) | Shanghai Chaori Solar Energy Science & Technology CRM290S156P-72(T) | Shanghai Chaori Solar Energy Science & Technology CRM295S156P-72(T) | Shanghai Chaori Solar Energy Science & Technology CRM300S156P-72(T) | Shanghai ST Solar STP190-48 | Shanghai ST Solar STP190-54 | Shanghai ST Solar STM195-72 | Shanghai ST Solar STP195-48 | Shanghai ST Solar STP195-54 | Shanghai ST Solar STM200-72 | Shanghai ST Solar STP200-48 | Shanghai ST Solar STP200-54 | Shanghai ST Solar STP205-54 | Shanghai ST Solar STM210-96 | Shanghai ST Solar STP210-54 | Shanghai ST Solar STP210-60 | Shanghai ST Solar STP215-54 | Shanghai ST Solar STP215-60 | Shanghai ST Solar STP220-54 | Shanghai ST Solar STP220-60 | Shanghai ST Solar STM225-96 | Shanghai ST Solar STP225-54 | Shanghai ST Solar STP225-60 | Shanghai ST Solar STP230-60 | Shanghai ST Solar STM235-96 | Shanghai ST Solar STP235-60 | Shanghai ST Solar STM240-96 | Shanghai ST Solar STP240-60 | Shanghai ST Solar STM245-96 | Shanghai ST Solar STP245-60 | Shanghai ST Solar STP245-72 | Shanghai ST Solar STM250-96 | Shanghai ST Solar STP250-60 | Shanghai ST Solar STP250-72 | Shanghai ST Solar STM255-104 | Shanghai ST Solar STM255-96 | Shanghai ST Solar STP255-72 | Shanghai ST Solar STM260-104 | Shanghai ST Solar STM260-96 | Shanghai ST Solar STP260-72 | Shanghai ST Solar STM265-104 | Shanghai ST Solar STP265-72 | Shanghai ST Solar STM270-104 | Shanghai ST Solar STP270-72 | Shanghai ST Solar STM275-104 | Shanghai ST Solar STP275-72 | Shanghai ST Solar STM280-104 | Shanghai ST Solar STP280-72 | Shanghai ST Solar STM285-104 | Shanghai ST Solar STP285-72 | Shanghai ST Solar STP290-72 | Shanghai ST Solar STP295-72 | Shanghai ST Solar STP300-72 | Shanghai ST Solar STM325-130 | Shanghai ST Solar STM330-130 | Shanghai ST Solar STM335-130 | Shanghai ST Solar STM340-130 | Shanghai ST Solar STM345-130 | Shanghai ST Solar STM350-130 | Shanghai Topsolar Green Energy TSM72-125M 160W | Shanghai Topsolar Green Energy TSM72-125M 165W | Shanghai Topsolar Green Energy TSM72-125M 170W | Shanghai Topsolar Green Energy TSM72-125M 175W | Shanghai Topsolar Green Energy TSM72-125M 180W | Shanghai Topsolar Green Energy TSM72-125M 185W | Shanghai Topsolar Green Energy TSM48-156M 190W | Shanghai Topsolar Green Energy TSM72-125M 190W | Shanghai Topsolar Green Energy TSM48-156M 195W | Shanghai Topsolar Green Energy TSM72-125M 195W | Shanghai Topsolar Green Energy TSM48-156M 200W | Shanghai Topsolar Green Energy TSM48-156M 205W | Shanghai Topsolar Green Energy TSM60-156M 210W | Shanghai Topsolar Green Energy TSM60-156M 235W | Shanghai Topsolar Green Energy TSM60-156M 240W | Shanghai Topsolar Green Energy TSM96-125M 240W | Shanghai Topsolar Green Energy TSM60-156M 245W | Shanghai Topsolar Green Energy TSM96-125M 245W | Shanghai Topsolar Green Energy TSM60-156M 250W | Shanghai Topsolar Green Energy TSM96-125M 250W | Shanghai Topsolar Green Energy TSM60-156M 255W | Shanghai Topsolar Green Energy TSM96-125M 255W | Shanghai Topsolar Green Energy TSM96-125M 260W | Shanghai Topsolar Green Energy TSM72-156M 280W | Shanghai Topsolar Green Energy TSM72-156M 285W | Shanghai Topsolar Green Energy TSM72-156M 290W | Shanghai Topsolar Green Energy TSM72-156M 295W | Shanghai Topsolar Green Energy TSM72-156M 300W | Shanghai Topsolar Green Energy TSM72-156M 305W | Shangpin Solar SPSM-175D | Shangpin Solar SPSM-180D | Shangpin Solar SPSM-185D | Shangpin Solar SPSM-215P | Shangpin Solar SPSM-220P | Shangpin Solar SPSM-225D | Shangpin Solar SPSM-225P | Shangpin Solar SPSM-230D | Shangpin Solar SPSM-230P | Shangpin Solar SPSM-235D | Shangpin Solar SPSM-235P | Shangpin Solar SPSM-240D | Shangpin Solar SPSM-245D | Shangpin Solar SPSM-260D | Shangpin Solar SPSM-265D | Shangpin Solar SPSM-270D | Shangpin Solar SPSM-275D | Shangpin Solar SPSM-280D | Shangpin Solar SPSM-285D | Shangpin Solar SPSM-290D | Sharp ND-62RU1 | Sharp ND-62RU1F | Sharp ND-62RU2 | Sharp ND-62RUC1 | Sharp ND-65RU1F | Sharp ND-65RUC1 | Sharp ND-72ELU | Sharp ND-72ELUC | Sharp ND-72ELUF | Sharp ND-72ERU | Sharp ND-72ERUC | Sharp ND-72ERUF | Sharp ND-V075CL | Sharp ND-V075CR | Sharp NA-V115H1 | Sharp NA-V121H1 | Sharp ND-123UJF | Sharp NA-V128H1 | Sharp ND-130UJF | Sharp NA-V135H1 | Sharp ND-N2ECU | Sharp ND-N2ECUC | Sharp ND-N2ECUF | Sharp NE-160U1 | Sharp ND-162U1F | Sharp ND-162U1Y | Sharp ND-162U2 | Sharp NE-165U1 | Sharp NE-165U5 | Sharp NE-165UC1 | Sharp ND-167U1 | Sharp ND-167U1F | Sharp ND-167U1Y | Sharp ND-167U2 | Sharp ND-167U3A | Sharp ND-167UC1 | Sharp NE-170U1 | Sharp NE-170UC1 | Sharp NT-170U1 | Sharp NT-170UC1 | Sharp NT-175U1 | Sharp NT-175UC1 | Sharp ND-176U1Y | Sharp ND-176UC1 | Sharp NT-180U1 | Sharp NU-U180FC | Sharp ND-181U1 | Sharp ND-181U1F | Sharp ND-181U2 | Sharp ND-187U1 | Sharp ND-187U1F | Sharp ND-187U2 | Sharp ND-187UC1 | Sharp ND-198U1F | Sharp ND-198UC1 | Sharp ND-200U1 | Sharp ND-200U1F | Sharp ND-200U2 | Sharp ND-200UC1 | Sharp ND-208U1 | Sharp ND-208U1F | Sharp ND-208U2 | Sharp ND-208UC1 | Sharp ND-208UCJ | Sharp NU-U208FC | Sharp ND-216QCJ | Sharp ND-216U1F | Sharp ND-216U2 | Sharp ND-216UC1 | Sharp ND-216UCJ | Sharp ND-U216C1 | Sharp ND-220U1F | Sharp ND-220UC1 | Sharp ND-220UCJ | Sharp ND-224QCJ | Sharp ND-224U1F | Sharp ND-224UC1 | Sharp ND-224UCJ | Sharp ND-U224C1 | Sharp ND-230QCJ | Sharp ND-230UC1 | Sharp ND-230UCJ | Sharp ND-F2Q230 | Sharp ND-H230Q2 | Sharp ND-L230Q1 | Sharp ND-L230Q2 | Sharp ND-Q230C5 | Sharp ND-Q230F4 | Sharp ND-Q230Q2 | Sharp ND-U230C1 | Sharp ND-U230Q1 | Sharp ND-U230Q2 | Sharp ND-V230A1 | Sharp NU-Q230F4 | Sharp NU-U230F3 | Sharp NU-U230F4 | Sharp ND-235QCJ | Sharp ND-F2Q235 | Sharp ND-H235Q2 | Sharp ND-L235Q1 | Sharp ND-L235Q2 | Sharp ND-Q235C5 | Sharp ND-Q235F4 | Sharp ND-Q235Q2 | Sharp ND-U235Q1 | Sharp ND-U235Q2 | Sharp NU-Q235F2 | Sharp NU-Q235F4 | Sharp NU-U235F1 | Sharp NU-U235F2 | Sharp NU-U235F3 | Sharp NU-U235F4 | Sharp ND-240QCJ | Sharp ND-F5Q240 | Sharp ND-H240Q2 | Sharp ND-L240Q2 | Sharp ND-Q240Q2 | Sharp ND-U240Q2 | Sharp NU-Q240F2 | Sharp NU-Q240W4 | Sharp NU-U240F1 | Sharp NU-U240F2 | Sharp NU-U240P1 | Sharp NU-U240P2 | Sharp ND-245QCJ | Sharp ND-245QCS | Sharp ND-F5Q245 | Sharp ND-H245Q2 | Sharp ND-L245Q2 | Sharp ND-Q245F7 | Sharp ND-Q245Q2 | Sharp ND-U245Q2 | Sharp NU-Q245F2 | Sharp NU-Q245W2 | Sharp NU-Q245W4 | Sharp NU-U245P1 | Sharp NU-U245P2 | Sharp ND-250QCS | Sharp ND-Q250F7 | Sharp NU-Q250W2 | Sharp NU-Q250W4 | Sharp ND-F4Q295 | Sharp ND-F4Q300 | Sharp NU-SC350 | Sharp NU-SC360 | Shenzhen Topray Solar TPS107S-175W(48) | Shenzhen Topray Solar TPS105S-180W(48) | Shenzhen Topray Solar TPS107S-180W(48) | Shenzhen Topray Solar TPS105S-185W(48) | Shenzhen Topray Solar TPS107S-185W(48) | Shenzhen Topray Solar TPS105S-190W(48) | Shenzhen Topray Solar TPS107S-190W(54) | Shenzhen Topray Solar TPS107S-195W(54) | Shenzhen Topray Solar TPS105S-200W(54) | Shenzhen Topray Solar TPS107S-200W(54) | Shenzhen Topray Solar TPS105S-205W(54) | Shenzhen Topray Solar TPS107S-205W(54) | Shenzhen Topray Solar TPS105S-210W(54) | Shenzhen Topray Solar TPS107S-210W(54) | Shenzhen Topray Solar TPS105S-215W(54) | Shenzhen Topray Solar TPS107S-215W(60) | Shenzhen Topray Solar TPS105S-220W(54) | Shenzhen Topray Solar TPS107S-220W(60) | Shenzhen Topray Solar TPS107S-225W(60) | Shenzhen Topray Solar TPS105S-230W(60) | Shenzhen Topray Solar TPS107S-230W(60) | Shenzhen Topray Solar TPS105S-235W(60) | Shenzhen Topray Solar TPS105S-240W(60) | Shenzhen Topray Solar TPS105S-245W(60) | Shenzhen Topray Solar TPS105S-250W(60) | Shenzhen Topray Solar TPS107S-260W(72) | Shenzhen Topray Solar TPS107S-265W(72) | Shenzhen Topray Solar TPS107S-270W(72) | Shenzhen Topray Solar TPS107S-275W(72) | Shenzhen Topray Solar TPS105S-280W(72) | Shenzhen Topray Solar TPS107S-280W(72) | Shenzhen Topray Solar TPS105S-285W(72) | Shenzhen Topray Solar TPS105S-290W(72) | Shenzhen Topray Solar TPS105S-295W(72) | Shenzhen Topray Solar TPS105S-300W(72) | Shenzhen Zhongjing Solar PWM-170W | Shenzhen Zhongjing Solar PWM-175W | Shenzhen Zhongjing Solar PWM-180W | Shenzhen Zhongjing Solar P6Y-230 | Shenzhen Zhongjing Solar P6Y-235 | Shenzhen Zhongjing Solar P6Y-240 | Shenzhen Zhongjing Solar P6Y-245 | Shenzhen Zhongjing Solar M9X-250 | Shenzhen Zhongjing Solar P6Y-250 | Shenzhen Zhongjing Solar M9X-255 | Shenzhen Zhongjing Solar M9X-260 | Shenzhen Zhongjing Solar M9X-265 | Shenzhen Zhongjing Solar P7Y-270 | Shenzhen Zhongjing Solar P7Y-275 | Shenzhen Zhongjing Solar P7Y-280 | Shenzhen Zhongjing Solar P7Y-285 | Shenzhen Zhongjing Solar P7Y-290 | Shinsung Solar Energy SS-BM245B3 | Shinsung Solar Energy SS-BM250B3 | Shinsung Solar Energy SS-BM255B3 | Shinsung Solar Energy SS-BM260B3 | Shinsung Solar Energy SS-BM265B3 | Shinsung Solar Energy SS-DM290B3 | Shinsung Solar Energy SS-DM295B3 | Shinsung Solar Energy SS-DM300B3 | Shinsung Solar Energy SS-DM305B3 | Shinsung Solar Energy SS-DM310B3 | Shinsung Solar Energy SS-DM315B3 | Shinsung Solar Energy SS-DM320B3 | Signet Solar S4 | Signet Solar S2 | Signet Solar S3 | Signet Solar S1 | Silevo Triex R215 | Silevo Triex R215 Black | Silevo Triex R220 | Silevo Triex R220 Black | Silevo Triex R225 | Silevo Triex R225 Black | Silevo Triex R230 | Silevo Triex R230 Black | Silevo Triex R235 | Silevo Triex R235 Black | Silevo Triex H60-270 | Silevo U270 | Silevo U270 Black | Silevo U275 | Silevo U275 Black | Silevo Triex H60-280 | Silevo Triex U-280 SleekBlack | Silevo U280 | Silevo U280 Black | Silevo Triex U-285 SleekBlack | Silevo W285-RB | Silevo Triex H60-290 | Silevo Triex U290 | Silevo Triex U290 Black | Silevo Triex U-290 SleekBlack | Silevo W290-RB | Silevo W290-RW | Silevo Triex U295 | Silevo Triex U295 Black | Silevo Triex U-295 SleekBlack | Silevo W295-RB | Silevo W295-RW | Silevo Triex U300 | Silevo Triex U300 Black | Silevo W300-RB | Silevo W300-RW | Silevo Triex U305 | Silevo Triex U305 Black | Silevo W305-RB | Silevo W305-RW | Silevo Triex U310 | Silevo Triex U310 Black | Silevo W310-RB | Silevo W310-RW | Silevo W315-RB | Silevo W315-RW | Silevo W320-RW | Silevo W325-RW | Silevo W330-RW | Silevo W335-RW | Silevo W340-RW | Silfab SLA240P | Silfab SLA245P | Silfab SSA245P | Silfab SLA250P | Silfab SSA250P | Silfab SLA255P | Silfab SSA255P | Silfab SLA260M | Silfab SLA260P | Silfab SSA260P | Silfab SLA265M | Silfab SLA265P | Silfab SSA265M | Silfab SSA265P | Silfab SLA270M | Silfab SSA270M | Silfab SLA275M | Silfab SSA275M | Silfab SLA280M | Silfab SSA280M | Silfab SLA285M | Silfab SLA290M | Silfab SLG290P | Silfab SSG290P | Silfab SLA295M | Silfab SLG295P | Silfab SSG295P | Silfab SLA300M | Silfab SLG300P | Silfab SSG300P | Silfab SLA305M | Silfab SLG305P | Silfab SSG305P | Silfab SLA310M | Silfab SLG310P | Silfab SSG310P | Silfab SLG315M | Silfab SLG315P | Silfab SSG315M | Silfab SSG315P | Silfab SLG320M | Silfab SLG320P | Silfab SSG320M | Silfab SSG320P | Silfab SLG325M | Silfab SSG325M | Silfab SLG330M | Silfab SSG330M | Silfab SLG335M | Silfab SLGX 335 Clear | Silfab SSG335M | Silfab SLGX 340 Clear | Silfab SLGX 340 White | Silfab SLG345M | Silfab SLGX 345 Clear | Silfab SLGX 345 White | Silfab SLG350M | Silfab SLGX 350 White | Silfab SLG360M | Silfab SLG365M | Silfab SLG370M | Silfab Solar SLG340M | Silfab Solar SLG355M | Silfab Solar Inc SLA-X 285 Clear | Silfab Solar Inc SLA-X 290 Clear | Silfab Solar Inc SLA-X 295 Clear | Silfab Solar Inc SLA-X 300 Clear | Silicon Energy SiE-165 | Silicon Energy SiE-170 | Silicon Energy SiE-175 | Silicon Energy SiE-180 | Silicon Energy SiE-185 | Silicon Energy SiE-190 | Silicon Energy SiE-195 | Silicon Energy SiE-200 | Silicon Energy SiE-205 | Silicon Energy SiE-210 | Silicon Energy SiE-215 | Silicon Energy SiE-220 | Silicon Energy SiE-V-275 | Silicon Energy SiE-V-280 | Silicon Energy SiE-V-285 | Siliken Canada SLK60P6L BLK/WHT 205Wp | Siliken Canada SLK60P6L SLV/WHT 205Wp | Siliken Canada SLK60P6L BLK/WHT 210Wp | Siliken Canada SLK60P6L SLV/WHT 210Wp | Siliken Canada SLK60P6L BLK/BLK 215Wp | Siliken Canada SLK60P6L BLK/WHT 215Wp | Siliken Canada SLK60P6L SLV/WHT 215Wp | Siliken Canada SLK60P6L BLK/BLK 220Wp | Siliken Canada SLK60P6L BLK/WHT 220Wp | Siliken Canada SLK60P6L SLV/WHT 220Wp | Siliken Canada SLK60P6L BLK/BLK 225Wp | Siliken Canada SLK60P6L BLK/WHT 225Wp | Siliken Canada SLK60P6L SLV/WHT 225Wp | Siliken Canada SLK60P6L BLK/BLK 230Wp | Siliken Canada SLK60P6L BLK/WHT 230Wp | Siliken Canada SLK60P6L SLV/WHT 230Wp | Siliken Canada SLK60P6L BLK/BLK 235Wp | Siliken Canada SLK60P6L BLK/WHT 235Wp | Siliken Canada SLK60P6L SLV/WHT 235Wp | Siliken Canada SLK60P6L BLK/BLK 240Wp | Siliken Canada SLK60P6L BLK/WHT 240Wp | Siliken Canada SLK60P6L SLV/WHT 240Wp | Siliken Canada SLK60P6L BLK/BLK 245Wp | Siliken Canada SLK60P6L BLK/WHT 245Wp | Siliken Canada SLK60P6L SLV/WHT 245Wp | Siliken Canada SLK60P6L BLK/BLK 250Wp | Siliken Canada SLK60P6L BLK/WHT 250Wp | Siliken Canada SLK60P6L SLV/WHT 250Wp | Siliken Canada SLK60P6L BLK/WHT 255Wp | Siliken Canada SLK60P6L SLV/WHT 255Wp | Siliken Canada SLK72P6L BLK/WHT 270Wp | Siliken Canada SLK72P6L SLV/WHT 270Wp | Siliken Canada SLK72P6L BLK/WHT 275Wp | Siliken Canada SLK72P6L SLV/WHT 275Wp | Siliken Canada SLK72P6L BLK/WHT 280Wp | Siliken Canada SLK72P6L SLV/WHT 280Wp | Siliken Canada SLK72P6L BLK/WHT 285Wp | Siliken Canada SLK72P6L SLV/WHT 285Wp | Siliken Canada SLK72P6L BLK/WHT 290Wp | Siliken Canada SLK72P6L SLV/WHT 290Wp | Siliken Canada SLK72P6L BLK/WHT 295Wp | Siliken Canada SLK72P6L SLV/WHT 295Wp | Siliken Canada SLK72P6L BLK/WHT 300Wp | Siliken Canada SLK72P6L SLV/WHT 300Wp | Siliken Canada SLK72P6L BLK/WHT 305Wp | Siliken Canada SLK72P6L SLV/WHT 305Wp | Siliken Manufacturing SLK72P6L 310Wp BLK/WHT | Siliken Manufacturing SLK72P6L 310Wp SLV/WHT | Siliken Manufacturing SLK72P6L 315Wp BLK/WHT | Siliken Manufacturing SLK72P6L 315Wp SLV/WHT | Siliken Manufacturing USA SLK60P6L BLK/WHT 205Wp | Siliken Manufacturing USA SLK60P6L SLV/WHT 205Wp | Siliken Manufacturing USA SLK60P6L BLK/WHT 210Wp | Siliken Manufacturing USA SLK60P6L SLV/WHT 210Wp | Siliken Manufacturing USA SLK60P6L BLK/BLK 215Wp | Siliken Manufacturing USA SLK60P6L BLK/WHT 215Wp | Siliken Manufacturing USA SLK60P6L SLV/WHT 215Wp | Siliken Manufacturing USA SLK60P6L BLK/BLK 220Wp | Siliken Manufacturing USA SLK60P6L BLK/WHT 220Wp | Siliken Manufacturing USA SLK60P6L SLV/WHT 220Wp | Siliken Manufacturing USA SLK60P6L BLK/BLK 225Wp | Siliken Manufacturing USA SLK60P6L BLK/WHT 225Wp | Siliken Manufacturing USA SLK60P6L SLV/WHT 225Wp | Siliken Manufacturing USA SLK60P6L BLK/BLK 230Wp | Siliken Manufacturing USA SLK60P6L BLK/WHT 230Wp | Siliken Manufacturing USA SLK60P6L SLV/WHT 230Wp | Siliken Manufacturing USA SLK60P6L BLK/BLK 235Wp | Siliken Manufacturing USA SLK60P6L BLK/WHT 235Wp | Siliken Manufacturing USA SLK60P6L SLV/WHT 235Wp | Siliken Manufacturing USA SLK60P6L BLK/BLK 240Wp | Siliken Manufacturing USA SLK60P6L BLK/WHT 240Wp | Siliken Manufacturing USA SLK60P6L SLV/WHT 240Wp | Siliken Manufacturing USA SLK60P6L BLK/BLK 245Wp | Siliken Manufacturing USA SLK60P6L BLK/WHT 245Wp | Siliken Manufacturing USA SLK60P6L SLV/WHT 245Wp | Siliken Manufacturing USA SLK60P6L BLK/BLK 250Wp | Siliken Manufacturing USA SLK60P6L BLK/WHT 250Wp | Siliken Manufacturing USA SLK60P6L SLV/WHT 250Wp | Siliken Manufacturing USA SLK60P6L BLK/WHT 255Wp | Siliken Manufacturing USA SLK60P6L SLV/WHT 255Wp | Siliken Manufacturing USA SLK72P6L BLK/WHT 270Wp | Siliken Manufacturing USA SLK72P6L SLV/WHT 270Wp | Siliken Manufacturing USA SLK72P6L BLK/WHT 275Wp | Siliken Manufacturing USA SLK72P6L SLV/WHT 275Wp | Siliken Manufacturing USA SLK72P6L BLK/WHT 280Wp | Siliken Manufacturing USA SLK72P6L SLV/WHT 280Wp | Siliken Manufacturing USA SLK72P6L BLK/WHT 285Wp | Siliken Manufacturing USA SLK72P6L SLV/WHT 285Wp | Siliken Manufacturing USA SLK72P6L BLK/WHT 290Wp | Siliken Manufacturing USA SLK72P6L SLV/WHT 290Wp | Siliken Manufacturing USA SLK72P6L BLK/WHT 295Wp | Siliken Manufacturing USA SLK72P6L SLV/WHT 295Wp | Siliken Manufacturing USA SLK72P6L BLK/WHT 300Wp | Siliken Manufacturing USA SLK72P6L SLV/WHT 300Wp | Siliken Manufacturing USA SLK72P6L BLK/WHT 305Wp | Siliken Manufacturing USA SLK72P6L SLV/WHT 305Wp | Siliken Manufacturing USA SLK72P6L 310Wp BLK/WHT | Siliken Manufacturing USA SLK72P6L 310Wp SLV/WHT | Siliken Manufacturing USA SLK72P6L 315Wp BLK/WHT | Siliken Manufacturing USA SLK72P6L 315Wp SLV/WHT | Siliken Modules SLK60P6L BLK/WHT 205Wp | Siliken Modules SLK60P6L SLV/WHT 205Wp | Siliken Modules SLK60P6L BLK/WHT 210Wp | Siliken Modules SLK60P6L SLV/WHT 210Wp | Siliken Modules SLK60P6L BLK/BLK 215Wp | Siliken Modules SLK60P6L BLK/WHT 215Wp | Siliken Modules SLK60P6L SLV/WHT 215Wp | Siliken Modules SLK60P6L BLK/BLK 220Wp | Siliken Modules SLK60P6L BLK/WHT 220Wp | Siliken Modules SLK60P6L SLV/WHT 220Wp | Siliken Modules SLK60P6L BLK/BLK 225Wp | Siliken Modules SLK60P6L BLK/WHT 225Wp | Siliken Modules SLK60P6L SLV/WHT 225Wp | Siliken Modules SLK60P6L BLK/BLK 230Wp | Siliken Modules SLK60P6L BLK/WHT 230Wp | Siliken Modules SLK60P6L SLV/WHT 230Wp | Siliken Modules SLK60P6L BLK/BLK 235Wp | Siliken Modules SLK60P6L BLK/WHT 235Wp | Siliken Modules SLK60P6L SLV/WHT 235Wp | Siliken Modules SLK60P6L BLK/BLK 240Wp | Siliken Modules SLK60P6L BLK/WHT 240Wp | Siliken Modules SLK60P6L SLV/WHT 240Wp | Siliken Modules SLK60P6L BLK/BLK 245Wp | Siliken Modules SLK60P6L BLK/WHT 245Wp | Siliken Modules SLK60P6L SLV/WHT 245Wp | Siliken Modules SLK60P6L BLK/BLK 250Wp | Siliken Modules SLK60P6L BLK/WHT 250Wp | Siliken Modules SLK60P6L SLV/WHT 250Wp | Siliken Modules SLK60P6L BLK/WHT 255Wp | Siliken Modules SLK60P6L SLV/WHT 255Wp | Siliken Modules SLK72P6L BLK/WHT 270Wp | Siliken Modules SLK72P6L SLV/WHT 270Wp | Siliken Modules SLK72P6L BLK/WHT 275Wp | Siliken Modules SLK72P6L SLV/WHT 275Wp | Siliken Modules SLK72P6L BLK/WHT 280Wp | Siliken Modules SLK72P6L SLV/WHT 280Wp | Siliken Modules SLK72P6L BLK/WHT 285Wp | Siliken Modules SLK72P6L SLV/WHT 285Wp | Siliken Modules SLK72P6L BLK/WHT 290Wp | Siliken Modules SLK72P6L SLV/WHT 290Wp | Siliken Modules SLK72P6L BLK/WHT 295Wp | Siliken Modules SLK72P6L SLV/WHT 295Wp | Siliken Modules SLK72P6L BLK/WHT 300Wp | Siliken Modules SLK72P6L SLV/WHT 300Wp | Siliken Modules SLK72P6L BLK/WHT 305Wp | Siliken Modules SLK72P6L SLV/WHT 305Wp | Silray SRMA-150WP | Silray SRMA-155WP | Silray SRMA-160WP | Silray SRMA-165WP | Silray SRMA-170WP | Silray API-175M | Silray SRAP-175G6M | Silray SRAP-175G6S | Silray SRMA-175WP | Silray API-180M | Silray SR-180 | Silray SRAP-180G6M | Silray SRAP-180G6S | Silray SRMA-180WP | Silray API-185M | Silray API-185M(72)-XH | Silray SRAP-185G6M | Silray SRAP-185G6S | Silray API-190M(72)-XH | Silray SRAP-190G6M | Silray SRAP-190G6S | Silray SRAP-195G6M | Silray SRAP-195G6S | Silray SRAP-200G6M | Silray SRAP-200G6S | Silray SRAP-205G6M | Silray SRAP-205G6S | Silray SRAP-210G6M | Silray SRAP-210G6S | Silray API-215M | Silray API-220P | Silray API-225M | Silray API-230P | Silray API-230P(60)-XH | Silray API-235M | Silray API-235P(60)-XH | Silray API-270P | Silray API-280M(72)-XH | Sintek Photronic STK-S6C2PE-A | Sintek Photronic STK-S6C1ME-A | Sintek Photronic STK-S6B1PE-A | Sintek Photronic STK-S6B1ME-A | SmartFlower Energy Technology GmbH SFE 155 | Smartflower Energy Technology GmbH SFE215 | Smartflower Energy Technology GmbH SFE225 | SMX Capital SMX185 | SMX Capital SMX230P | SMX Capital SMX250P | SMX Capital SMX255P | SMX Capital SMX260P | Solar Enertech (Shanghai) SE175-72M | Solar Enertech (Shanghai) SE180-72M | Solar Enertech (Shanghai) SE185-72M | Solar Enertech (Shanghai) SE195-54P | Solar Enertech (Shanghai) SE200-54P | Solar Enertech (Shanghai) SE205-54P | Solar Enertech (Shanghai) SE210-54P | Solar Frontier SC70-US-P | Solar Frontier SF70-US-B | Solar Frontier SF70-US-P | Solar Frontier SC75-US-P | Solar Frontier SF75-US-B | Solar Frontier SF75-US-P | Solar Frontier SC80-US-P | Solar Frontier SF80-US-B | Solar Frontier SF80-US-P | Solar Frontier SF85-US-B | Solar Frontier SF85-US-P | Solar Frontier SF90-US-B | Solar Frontier SF130-L | Solar Frontier SF130-S | Solar Frontier SF130-S-1500 | Solar Frontier SF135-L | Solar Frontier SF135-S | Solar Frontier SF135-S-1500 | Solar Frontier SF140-L | Solar Frontier SF140-S | Solar Frontier SF140-S-1500 | Solar Frontier SF145-L | Solar Frontier SF145-S | Solar Frontier SF145-S-1500 | Solar Frontier SF150-L | Solar Frontier SF150-S | Solar Frontier SF150-S-1500 | Solar Frontier SF155-L | Solar Frontier SF155-S | Solar Frontier SF155-S-1500 | Solar Frontier SF160-S | Solar Frontier SF160-S-1500 | Solar Frontier SF165-S | Solar Frontier SF165-S-1500 | Solar Frontier SF170-S | Solar Frontier SF170-S-1500 | Solar Frontier SF175-S | Solar Frontier SF175-S-1500 | Solar Liberty SLX120P6-18 | Solar Liberty SLX125P6-18 | Solar Liberty SLX130P6-18 | Solar Liberty SLX135P6-18 | Solar Liberty SLX140P6-18 | Solar Liberty SLX200P6-30 | Solar Liberty SLX205P6-30 | Solar Liberty SLX210P6-30 | Solar Liberty SLX215P6-30 | Solar Liberty SLX220P6-30 | Solar Liberty SLX225P6-30 | Solar Liberty SLX230P6-30 | Solar Liberty SLX 235 USB | Solar Liberty SLX 235 USC | Solar Liberty SLX 235 USD | Solar Liberty SLX235P6-30 | Solar Liberty SLX 240 USB | Solar Liberty SLX 240 USC | Solar Liberty SLX 240 USD | Solar Liberty SLX240P6-36 | Solar Liberty SLX 245 USB | Solar Liberty SLX 245 USC | Solar Liberty SLX245P6-36 | Solar Liberty SLX 250 USB | Solar Liberty SLX 250 USC | Solar Liberty SLX 250 USD | Solar Liberty SLX250P6-36 | Solar Liberty SLX 255 USB | Solar Liberty SLX 255 USC | Solar Liberty SLX 255 USD | Solar Liberty SLX255P6-36 | Solar Liberty SLX 260 USB | Solar Liberty SLX 260 USC | Solar Liberty SLX 260 USD | Solar Liberty SLX260P6-36 | Solar Liberty SLX 265 USB | Solar Liberty SLX 265 USC | Solar Liberty SLX 265 USD | Solar Liberty SLX 265 USMB | Solar Liberty SLX 265 USMC | Solar Liberty SLX 265 USMD | Solar Liberty SLX265P6-36 | Solar Liberty SLX 270 USB | Solar Liberty SLX 270 USC | Solar Liberty SLX 270 USD | Solar Liberty SLX 270 USMC | Solar Liberty SLX 270 USMD | Solar Liberty SLX270P6-36 | Solar Liberty SLX275P6-36 | Solar Liberty SLX280P6-36 | Solar Liberty SLX285P6-36 | Solar Liberty SLX 290 USMC | Solar Liberty SLX 290 USMD | Solar Liberty SLX 295 USMC | Solar Liberty SLX 295 USMD | Solar Liberty SLX 300 USMC | Solar Liberty SLX 300 USMD | Solar Liberty SLX 305 USMC | Solar Liberty SLX 305 USMD | Solar Liberty SLX 310 USC | Solar Liberty SLX 310 USMC | Solar Liberty SLX 310 USMD | Solar Liberty SLX 315 USMC | Solar Liberty SLX 315 USMD | Solar Liberty SLX 320 USC | Solar Liberty SLX 320 USMC | Solar Liberty SLX 320 USMD | Solar Liberty SLX 325 USC | Solar Liberty SLX 325 USMC | Solar Liberty SLX 325 USMD | Solar Liberty SLX 330 USC | Solar Liberty SLX 330 USMC | Solar Liberty SLX 330 USMD | Solar Power (SPI) SP165FM52 | Solar Power (SPI) SP170FM12 | Solar Power (SPI) SP170FM22 | Solar Power (SPI) SP170FM52 | Solar Power (SPI) SP175FM12 | Solar Power (SPI) SP175FM52 | Solar Power (SPI) SP180FM12 | Solar Power (SPI) SP180FM52 | Solar Power (SPI) SP190FM52 | Solar Power (SPI) SP190FP12 | Solar Power (SPI) SP190FP52 | Solar Power (SPI) SP195FM12 | Solar Power (SPI) SP195FM52 | Solar Power (SPI) SP195FP12 | Solar Power (SPI) SP195FP42 | Solar Power (SPI) SP195FP52 | Solar Power (SPI) SP195FP82 | Solar Power (SPI) ES200PCFW | Solar Power (SPI) SP200FM12 | Solar Power (SPI) SP200FM52 | Solar Power (SPI) SP200FP12 | Solar Power (SPI) SP200FP42 | Solar Power (SPI) SP200FP52 | Solar Power (SPI) SP200FP82 | Solar Power (SPI) SP200FPA2 | Solar Power (SPI) SP200FPB2-01 | Solar Power (SPI) ES205PCFW | Solar Power (SPI) SP205FM12 | Solar Power (SPI) SP205FM52 | Solar Power (SPI) SP205FP12 | Solar Power (SPI) SP205FP42 | Solar Power (SPI) SP205FP52 | Solar Power (SPI) SP205FP82 | Solar Power (SPI) SP205FPA2 | Solar Power (SPI) SP205FPB2-01 | Solar Power (SPI) ES210PCFW | Solar Power (SPI) SP210FM12 | Solar Power (SPI) SP210FM52 | Solar Power (SPI) SP210FP12 | Solar Power (SPI) SP210FP42 | Solar Power (SPI) SP210FP52 | Solar Power (SPI) SP210FP82 | Solar Power (SPI) SP210FPA2 | Solar Power (SPI) SP210FPB2-01 | Solar Power (SPI) ES215PCFW | Solar Power (SPI) SP220FP12 | Solar Power (SPI) SP220FP52 | Solar Power (SPI) SP220FP82 | Solar Power (SPI) SP220FPA2 | Solar Power (SPI) SP220FPA2-02 | Solar Power (SPI) SP220FPB2-01 | Solar Power (SPI) SP225FP12 | Solar Power (SPI) SP225FP52 | Solar Power (SPI) SP225FP82 | Solar Power (SPI) SP225FPA2 | Solar Power (SPI) SP225FPA2-02 | Solar Power (SPI) SP225FPB2-01 | Solar Power (SPI) SP230FP12 | Solar Power (SPI) SP230FP52 | Solar Power (SPI) SP230FP82 | Solar Power (SPI) SP230FPA2 | Solar Power (SPI) SP230FPA2-02 | Solar Power (SPI) SP230FPB2-0 | Solar Power (SPI) SP230FPC2 | Solar Power (SPI) SP235FPA2-02 | Solar Power (SPI) SP235FPB2-01 | Solar Power (SPI) SP235FPC2 | Solar Power (SPI) SP240FPB2-01 | Solar Power (SPI) SP240FPC2 | Solar Power (SPI) ES245PABB | Solar Power (SPI) ES245PABW | Solar Power (SPI) ES245PAFB | Solar Power (SPI) ES245PAFW | Solar Power (SPI) SP245FPB2-01 | Solar Power (SPI) ES250PABB | Solar Power (SPI) ES250PABW | Solar Power (SPI) ES250PAFB | Solar Power (SPI) ES250PAFW | Solar Power (SPI) ES255PABB | Solar Power (SPI) ES255PABW | Solar Power (SPI) ES255PAFB | Solar Power (SPI) ES255PAFW | Solar Power (SPI) ES260PABB | Solar Power (SPI) ES260PABW | Solar Power (SPI) ES260PAFB | Solar Power (SPI) ES260PAFW | Solar Power (SPI) ES265PAFW | Solar Power (SPI) ES300PBFW | Solar Power (SPI) ES305PBFW | Solar Power (SPI) ES310PBFW | Solar Power (SPI) ES315PBFW | Solar Power (SPI) ES320PBFW | Solar Power Industries SPI-M160-60 | Solar Power Industries SPI-M170-60 | Solar Power Industries SPI-M180-60 | Solar Power Industries SPI-M190-60 | Solar Power Industries SPI-156-200W | Solar Power Industries SPI-M200-60 | Solar Power Industries SPI-M210-60 | Solar Power Industries SPI-M215-60 | Solar Power Industries SPI-M220-60 | Solar Power Industries SPI-M220W-60IM | Solar Power Industries SPI-M225-60 | Solar Power Industries SPI-M230-60 | Solar Power Industries SPI-M230W-60IM | Solar Power Industries SPI-M240W-60IM | Solar Semiconductor SSI-S6-125 | Solar Semiconductor SSI-S6-130 | Solar Semiconductor SSI-S6-135 | Solar Semiconductor SSI-S6-140 | Solar Semiconductor SSI-S6-145 | Solar Semiconductor SSI-S6-170 | Solar Semiconductor SSI-S6-175 | Solar Semiconductor SSI-S6-180 | Solar Semiconductor SSI-S6-185 | Solar Semiconductor SSI-S6-190 | Solar Semiconductor SSI-S6-195 | Solar Semiconductor SSI-S6-200 | Solar Semiconductor SSI-S6-205 | Solar Semiconductor SSI-S6-210 | Solar Semiconductor SSI-3M6-215 | Solar Semiconductor SSI-M6-215 | Solar Semiconductor SSI-S6-215 | Solar Semiconductor SSI-3M6-220 | Solar Semiconductor SSI-M6-220 | Solar Semiconductor SSI-S6-220 | Solar Semiconductor SSI-3M6-225 | Solar Semiconductor SSI-M6-225 | Solar Semiconductor SSI-S6-225 | Solar Semiconductor SSI-3M6-230 | Solar Semiconductor SSI-M6-230 | Solar Semiconductor SSI-S6-230 | Solar Semiconductor SSI-3M6-235 | Solar Semiconductor SSI-M6-235 | Solar Semiconductor SSI-S6-235 | Solar Semiconductor SSI-S6-260 | Solar Semiconductor SSI-S6-265 | Solar Semiconductor SSI-S6-270 | Solar Semiconductor SSI-S6-275 | Solar Semiconductor SSI-S6-280 | Solarbest Energy-Tech (Zhejiang) SE-M170(125) | Solarbest Energy-Tech (Zhejiang) ZSB-M170(125) | Solarbest Energy-Tech (Zhejiang) SE-M175(125) | Solarbest Energy-Tech (Zhejiang) ZSB-M175(125) | Solarbest Energy-Tech (Zhejiang) SE-M180(125) | Solarbest Energy-Tech (Zhejiang) ZSB-M180(125) | Solarbest Energy-Tech (Zhejiang) SE-M185(125) | Solarbest Energy-Tech (Zhejiang) ZSB-M185(125) | Solarbest Energy-Tech (Zhejiang) SE-M190(125) | Solarbest Energy-Tech (Zhejiang) ZSB-M190(125) | Solarbest Energy-Tech (Zhejiang) SE-M195(125) | Solarbest Energy-Tech (Zhejiang) ZSB-M195(125) | Solarbest Energy-Tech (Zhejiang) SE-M200(125) | Solarbest Energy-Tech (Zhejiang) ZSB-M200(125) | Solarbest Energy-Tech (Zhejiang) SE-M205(125) | Solarbest Energy-Tech (Zhejiang) ZSB-M205(125) | Solarbest Energy-Tech (Zhejiang) SE-M220(125) | Solarbest Energy-Tech (Zhejiang) SE-M220(156) | Solarbest Energy-Tech (Zhejiang) SE-P220(156) | Solarbest Energy-Tech (Zhejiang) ZSB-M220(125) | Solarbest Energy-Tech (Zhejiang) ZSB-M220(156) | Solarbest Energy-Tech (Zhejiang) ZSB-P220(156) | Solarbest Energy-Tech (Zhejiang) SE-M225(125) | Solarbest Energy-Tech (Zhejiang) SE-M225(156) | Solarbest Energy-Tech (Zhejiang) SE-P225(156) | Solarbest Energy-Tech (Zhejiang) ZSB-M225(125) | Solarbest Energy-Tech (Zhejiang) ZSB-M225(156) | Solarbest Energy-Tech (Zhejiang) ZSB-P225(156) | Solarbest Energy-Tech (Zhejiang) SE-M230(125) | Solarbest Energy-Tech (Zhejiang) SE-M230(156) | Solarbest Energy-Tech (Zhejiang) SE-P230(156) | Solarbest Energy-Tech (Zhejiang) ZSB-M230(125) | Solarbest Energy-Tech (Zhejiang) ZSB-M230(156) | Solarbest Energy-Tech (Zhejiang) ZSB-P230(156) | Solarbest Energy-Tech (Zhejiang) SE-M235(125) | Solarbest Energy-Tech (Zhejiang) SE-M235(156) | Solarbest Energy-Tech (Zhejiang) SE-P235(156) | Solarbest Energy-Tech (Zhejiang) ZSB-M235(125) | Solarbest Energy-Tech (Zhejiang) ZSB-M235(156) | Solarbest Energy-Tech (Zhejiang) ZSB-P235(156) | Solarbest Energy-Tech (Zhejiang) SE-M240(125) | Solarbest Energy-Tech (Zhejiang) SE-M240(156) | Solarbest Energy-Tech (Zhejiang) SE-P240(156) | Solarbest Energy-Tech (Zhejiang) ZSB-M240(125) | Solarbest Energy-Tech (Zhejiang) ZSB-M240(156) | Solarbest Energy-Tech (Zhejiang) ZSB-P240(156) | Solarbest Energy-Tech (Zhejiang) SE-M245(125) | Solarbest Energy-Tech (Zhejiang) SE-M245(156) | Solarbest Energy-Tech (Zhejiang) SE-P245(156) | Solarbest Energy-Tech (Zhejiang) ZSB-M245(125) | Solarbest Energy-Tech (Zhejiang) ZSB-M245(156) | Solarbest Energy-Tech (Zhejiang) ZSB-P245(156) | Solarbest Energy-Tech (Zhejiang) SE-M250(125) | Solarbest Energy-Tech (Zhejiang) SE-M250(156) | Solarbest Energy-Tech (Zhejiang) SE-P250(156) | Solarbest Energy-Tech (Zhejiang) ZSB-M250(125) | Solarbest Energy-Tech (Zhejiang) ZSB-M250(156) | Solarbest Energy-Tech (Zhejiang) ZSB-P250(156) | Solarbest Energy-Tech (Zhejiang) SE-M255(125) | Solarbest Energy-Tech (Zhejiang) SE-M255(156) | Solarbest Energy-Tech (Zhejiang) SE-P255(156) | Solarbest Energy-Tech (Zhejiang) ZSB-M255(125) | Solarbest Energy-Tech (Zhejiang) ZSB-M255(156) | Solarbest Energy-Tech (Zhejiang) ZSB-P255(156) | Solarbest Energy-Tech (Zhejiang) SE-M260(125) | Solarbest Energy-Tech (Zhejiang) SE-M260(156) | Solarbest Energy-Tech (Zhejiang) SE-P260(156) | Solarbest Energy-Tech (Zhejiang) ZSB-M260(125) | Solarbest Energy-Tech (Zhejiang) ZSB-M260(156) | Solarbest Energy-Tech (Zhejiang) ZSB-P260(156) | Solarbest Energy-Tech (Zhejiang) SE-M265(125) | Solarbest Energy-Tech (Zhejiang) SE-M265(156) | Solarbest Energy-Tech (Zhejiang) SE-P265(156) | Solarbest Energy-Tech (Zhejiang) ZSB-M265(125) | Solarbest Energy-Tech (Zhejiang) ZSB-M265(156) | Solarbest Energy-Tech (Zhejiang) ZSB-P265(156) | Solarbest Energy-Tech (Zhejiang) SE-M270(125) | Solarbest Energy-Tech (Zhejiang) SE-M270(156) | Solarbest Energy-Tech (Zhejiang) SE-P270(156) | Solarbest Energy-Tech (Zhejiang) ZSB-M270(125) | Solarbest Energy-Tech (Zhejiang) ZSB-M270(156) | Solarbest Energy-Tech (Zhejiang) ZSB-P270(156) | Solarbest Energy-Tech (Zhejiang) SE-M275(156) | Solarbest Energy-Tech (Zhejiang) SE-P275(156) | Solarbest Energy-Tech (Zhejiang) ZSB-M275(156) | Solarbest Energy-Tech (Zhejiang) ZSB-P275(156) | Solarbest Energy-Tech (Zhejiang) SE-M280(156) | Solarbest Energy-Tech (Zhejiang) SE-P280(156) | Solarbest Energy-Tech (Zhejiang) ZSB-M280(156) | Solarbest Energy-Tech (Zhejiang) ZSB-P280(156) | Solarbest Energy-Tech (Zhejiang) SE-M285(156) | Solarbest Energy-Tech (Zhejiang) SE-P285(156) | Solarbest Energy-Tech (Zhejiang) ZSB-M285(156) | Solarbest Energy-Tech (Zhejiang) ZSB-P285(156) | Solarbest Energy-Tech (Zhejiang) SE-M290(156) | Solarbest Energy-Tech (Zhejiang) SE-P290(156) | Solarbest Energy-Tech (Zhejiang) ZSB-M290(156) | Solarbest Energy-Tech (Zhejiang) ZSB-P290(156) | Solarbest Energy-Tech (Zhejiang) SE-M295(156) | Solarbest Energy-Tech (Zhejiang) SE-P295(156) | Solarbest Energy-Tech (Zhejiang) ZSB-M295(156) | Solarbest Energy-Tech (Zhejiang) ZSB-P295(156) | Solarbest Energy-Tech (Zhejiang) SE-M300(156) | Solarbest Energy-Tech (Zhejiang) SE-P300(156) | Solarbest Energy-Tech (Zhejiang) ZSB-M300(156) | Solarbest Energy-Tech (Zhejiang) ZSB-P300(156) | Solarbest Energy-Tech (Zhejiang) SE-M305(156) | Solarbest Energy-Tech (Zhejiang) SE-P305(156) | Solarbest Energy-Tech (Zhejiang) ZSB-M305(156) | Solarbest Energy-Tech (Zhejiang) ZSB-P305(156) | Solarbest Energy-Tech (Zhejiang) SE-P310(156) | Solarbest Energy-Tech (Zhejiang) ZSB-P310(156) | Solarbine SB-S240TA1 | Solarbine SB-S245TA1 | Solarbine SB-S250TA1 | Solarbine S6T AC | Solarbine SB-S255TA1 | Solarbine SB-S260TA1 | Solarbine SB-S360TA1 | Solarbine SB-M365NA1 | Solarbine SB-S365TA1 | Solarbine SB-M370NA1 | Solarbine SB-S370TA1 | Solarbine SB-M375NA1 | Solarbine SB-S375TA1 | Solarbine SB-M380NA1 | Solarbine SB-S380SA1 | Solarbine SB-S380TA1 | Solarbine SB-M385NA1 | Solarbine SB-S385SA1 | Solarbine SB-S385TA1 | Solarbine SB-M390NA1 | Solarbine SB-S390SA1 | Solarbine SB-S390TA1 | Solarbine SB-M395NA1 | Solarbine SB-S395SA1 | Solarbine SB-S400SA1 | Solarbine SB-S405SA1 | Solarbine SB-S410SA1 | Solarbine SB-S415SA1 | Solarbine SB-S420SA1 | SolarBridge Technologies SBT250-NA208/240-A121 | SolarBridge Technologies SBT250-NA208/240-A321 | SolarBridge Technologies SBT250-NA240-A111 | SolarBridge Technologies SBT250-NA240-A311 | SolarCity SC255 | SolarCity SC260 | SolarCity SC265 | SolarCity SC270 | SolarCity SC320 | SolarCity SC325 | SolarCity SC330 | SolarCity Corp SC310B2 | SolarCity Corp SC315B1 | SolarCity Corp SC315B2 | SolarCity Corp SC320B1 | Solarfennel PS6A-230 | Solarfennel PS6A-235 | Solarfennel PS6A-240 | Solarfennel PS6A-245 | Solarfennel MS9A-250 | Solarfennel PS6A-250 | Solarfennel MS9A-255 | Solarfennel MS9A-260 | Solarfennel MS9A-265 | Solarfennel PS7A-270 | Solarfennel PS7A-275 | Solarfennel PS7A-280 | Solarfennel PS7A-285 | Solarfennel PS7A-290 | Solarfun Power SF220-30-P230 | Solarfun Power SF220-30-P235 | Solarfun Power SF220-30-P240 | Solargate Technology SG-2150 | Solargate Technology SG-2200 | Solargate Technology SG-2250 | Solargate Technology SG-2300 | Solargate Technology SG-2350 | Solaria Corporation Solaria 210 | Solaria Corporation Solaria 210 Frameless | Solaria Corporation Solaria 220 | Solaria Corporation Solaria 220 Frameless | Solaria Corporation Solaria 225 | Solaria Corporation Solaria 225 Frameless | Solaria Corporation Solaria 230 | Solaria Corporation Solaria 230 Frameless | Solaria Corporation Solaria 250 | Solaria Corporation Solaria 255 | Solaria Corporation Solaria 260 | Solaria Corporation Solaria 265 | Solaria Corporation Solaria 270 | Solaria Corporation Solaria 275 | Solaria Corporation Solaria 280 | Solaria Corporation Solaria PowerXT-320R-PX | Solaria Corporation Solaria PowerXT-325R-PX | Solaria Corporation Solaria PowerXT-330R-BX | Solaria Corporation Solaria PowerXT-335R-PD | Solaria Corporation Solaria PowerXT-335R-PX | Solaria Corporation Solaria PowerXT-340R-BD | Solaria Corporation Solaria PowerXT-340R-PD | Solaria Corporation Solaria PowerXT-345R-BD | Solaria Corporation Solaria PowerXT-345R-PD | Solaria Corporation Solaria PowerXT-350R-AC | Solaria Corporation Solaria PowerXT-350R-BD | Solaria Corporation Solaria PowerXT-350R-PD | Solaria Corporation Solaria PowerXT-360R-AC | Solaria Corporation Solaria PowerXT-360R-PD | Solaria Corporation Solaria PowerXT-U-360 | Solaria Corporation Solaria PowerXT-U-365 | Solaria Corporation Solaria PowerXT-U-370 | Solaria Corporation Solaria PowerXT-400C-WX | Solaria Corporation Solaria PowerXT-400U-WX | Solaria Corporation Solaria PowerXT-405C-WX | Solaria Corporation Solaria PowerXT-405U-WX | Solaria Corporation Solaria PowerXT-420C-BD | Solaria Corporation Solaria PowerXT-430C-PD | Solaria Corporation Solaria PowerXT-440C-PD | Solarland USA SLP115S-17H | Solarland USA SLP120S-17H | Solarland USA SLP125S-17H | Solarland USA SLP160S-24H | Solarland USA SLP165S-24H | Solarland USA SLP170S-24H | Solarland USA SLP175S-24H | Solarland USA SLP175S-24J | Solarland USA SLP180S-24H | Solarland USA SLP180S-24J | Solarland USA SLP185S-24H | Solarland USA SLP185S-24J | Solarland USA SLP185S-72 | Solarland USA SLP190S-24H | Solarland USA SLP190S-72 | Solarland USA SLP195S-24H | Solarland USA SLP200-18H | Solarland USA SLP200S-24H | Solarland USA SLP205-18H | Solarland USA SLP210-18H | Solarland USA SLP215-18H | Solarland USA SLP215-60 | Solarland USA SLP220-18H | Solarland USA SLP220-60 | Solarland USA SLP225-60 | Solarland USA SLP230-18H | Solarland USA SLP230-60 | Solarland USA SLP230S-96 | Solarland USA SLP235-18H | Solarland USA SLP235-60 | Solarland USA SLP240-18H | Solarland USA SLP240S-96 | Solarland USA SLP245S-96 | Solarland USA SLP250S-96 | Solarmax SEAP60-230 | Solarmax SEAP60-235 | Solarmax SEAP60-240 | Solarmax SEAP60-245 | Solarmax SEAP60-250 | Solarmax SMXUSA250 | Solarmax SEAP60-255 | Solarmax SEAP60-260 | Solarmax SMXUSA260 | Solarmax SEAP72-280 | Solarmax SEAP72-285 | Solarmax SEAP72-290 | Solarmax SEAP72-295 | Solarmax SEAP72-300 | Solarmax SEAP72-305 | SolarPark Korea SPP 220 | SolarPark Korea SPP 225 | SolarPark Korea SPP 230 | SolarPark Korea SPP235 | SolarPark Korea SPP240 | SolarPark Korea SPP245 | SolarPark Korea SPP245 mono | SolarPark Korea SPP 250 | SolarPark Korea SPP250 mono | SolarPark Korea SPP255 mono | SolarPark Korea SPP260 mono | Solarpeace P6Y-230 | Solarpeace P6Y-235 | Solarpeace P6Y-240 | Solarpeace P6Y-245 | Solarpeace M9X-250 | Solarpeace P6Y-250 | Solarpeace M9X-255 | Solarpeace M9X-260 | Solarpeace M9X-265 | Solarpeace P7Y-270 | Solarpeace P7Y-275 | Solarpeace P7Y-280 | Solarpeace P7Y-285 | Solarpeace P7Y-290 | Solartec S72MC-190 | Solartec S72MC-195 | Solartec S72MC-200 | Solartec S72MC-205 | Solartec S72MC-210 | Solartec S60MC-245 | Solartec S60MC-250 | Solartec S60MC-255 | Solartec S60MC-260 | Solartec S72PC-270 | Solartec S72PC-275 | Solartec S72PC-280 | Solartec S72PC-285 | Solartec S72MC6-290 | Solartec S72PC-290 | Solartec S72MC6-295 | Solartec S72PC-295 | Solartec S72MC6-300 | Solartec S72PC-300 | Solartec S72MC6-305 | Solartec S72PC-305 | Solartec S72MC6-310 | Solartec S72PC-310 | Solartec S72MC6-315 | Solartec S72PC-315 | Solartec S72MC6-320 | Solartec S72PC-320 | Solartec USA SDM-170/(165)-72M | Solartec USA SDM-170/(170)-72M | Solartec USA SDM-170/(175)-72M | Solartec USA SDM-170/(180)-72M | Solartec USA SDM-170/(185)-72M | Solartech Energy ASC-6P-36-130 | Solartech Energy ASC-6P-36-135 | Solartech Energy ASC-6P-36-140 | Solartech Energy ASC-6P-36-145 | Solartech Energy ASC-6P-36-150 | Solartech Energy ASC-6P-48-175 | Solartech Energy ASC-6P-48-180 | Solartech Energy ASC-6P-48-185 | Solartech Energy ASC-6P-48-190 | Solartech Energy ASC-6P-48-195 | Solartech Energy ASC-6P-48-200 | Solartech Energy ASC-6P-54-200 | Solartech Energy ASC-6P-54-205 | Solartech Energy ASC-6P-54-210 | Solartech Energy SEC-210W-M6-G | Solartech Energy ASC-6P-54-215 | Solartech Energy SEC-215W-M6-G | Solartech Energy ASC-6P-54-220 | Solartech Energy ASC-6P-60-220 | Solartech Energy SEC-220W-M6-G | Solartech Energy SEC-6P-60-220 | Solartech Energy ASC-6P-54-225 | Solartech Energy ASC-6P-60-225 | Solartech Energy ASC-6P-60-225-3BB | Solartech Energy SEC-225W-M6-G | Solartech Energy SEC-6P-60-225 | Solartech Energy ASC-6M-60-230-3BB | Solartech Energy ASC-6P-54-230 | Solartech Energy ASC-6P-60-230 | Solartech Energy ASC-6P-60-230-3BB | Solartech Energy SEC-230W-M6-G | Solartech Energy SEC-6P-60-230 | Solartech Energy ASC-6M-60-235-3BB | Solartech Energy ASC-6P-60-235 | Solartech Energy ASC-6P-60-235-3BB | Solartech Energy SEC-6P-60-235 | Solartech Energy ASC-6M-60-240-3BB | Solartech Energy ASC-6P-60-240 | Solartech Energy ASC-6P-60-240-3BB | Solartech Energy SEC-6P-60-240 | Solartech Energy ASC-6M-60-245-3BB | Solartech Energy ASC-6P-60-245 | Solartech Energy ASC-6P-60-245-3BB | Solartech Energy SEC-6P-60-245 | Solartech Energy ASC-6M-60-250-3BB | Solartech Energy ASC-6P-60-250 | Solartech Energy ASC-6P-60-250-3BB | Solartech Energy ASC-6M-60-255-3BB | Solartech Energy ASC-6P-60-255 | Solartech Energy ASC-6P-60-255-3BB | Solartech Energy ASC-6P-60A-255-3BB | Solartech Energy ASC-6M-60-260-3BB | Solartech Energy ASC-6P-60-260-3BB | Solartech Energy ASC-6P-60A-260-3BB | Solartech Energy ASC-6M-60-265-3BB | Solartech Energy ASC-6M-60A-265-3BB | Solartech Energy ASC-6P-60-265-3BB | Solartech Energy ASC-6P-60A-265-3BB | Solartech Energy ASC-6P-72-265 | Solartech Energy ASC-6M-60-270-3BB | Solartech Energy ASC-6M-60A-270-3BB | Solartech Energy ASC-6P-60-270-3BB | Solartech Energy ASC-6P-60A-270-3BB | Solartech Energy ASC-6P-72-270 | Solartech Energy ASC-6M-60-275-3BB | Solartech Energy ASC-6M-60A-275-3BB | Solartech Energy ASC-6P-72-275 | Solartech Energy ASC-6P-72-280 | Solartech Energy ASC-6P-72-280-3BB | Solartech Energy ASC-6M-72-285-3BB | Solartech Energy ASC-6P-72-285 | Solartech Energy ASC-6P-72-285-3BB | Solartech Energy ASC-6M-72-290-3BB | Solartech Energy ASC-6P-72-290 | Solartech Energy ASC-6P-72-290-3BB | Solartech Energy ASC-6M-72-295-3BB | Solartech Energy ASC-6P-72-295 | Solartech Energy ASC-6P-72-295-3BB | Solartech Energy ASC-6M-72-300-3BB | Solartech Energy ASC-6P-72-300 | Solartech Energy ASC-6P-72-300-3BB | Solartech Energy ASC-6M-72-305-3BB | Solartech Energy ASC-6P-72-305 | Solartech Energy ASC-6P-72-305-3BB | Solartech Energy ASC-6P-72B-305-3BB | Solartech Energy ASC-6P-72C-305-3BB | Solartech Energy ASC-6M-72-310-3BB | Solartech Energy ASC-6P-72-310-3BB | Solartech Energy ASC-6P-72B-310-3BB | Solartech Energy ASC-6P-72C-310-3BB | Solartech Energy ASC-6M-72-315-3BB | Solartech Energy ASC-6P-72-315-3BB | Solartech Energy ASC-6P-72B-315-3BB | Solartech Energy ASC-6P-72C-315-3BB | Solartech Energy ASC-6M-72-320-3BB | Solartech Energy ASC-6M-72B-320-3BB | Solartech Energy ASC-6M-72C-320-3BB | Solartech Energy ASC-6P-72-320-3BB | Solartech Energy ASC-6P-72B-320-3BB | Solartech Energy ASC-6P-72C-320-3BB | Solartech Energy ASC-6M-72-325-3BB | Solartech Energy ASC-6M-72B-325-3BB | Solartech Energy ASC-6M-72C-325-3BB | Solartech Energy ASC-6P-72-325-3BB | Solartech Energy ASC-6P-72B-325-3BB | Solartech Energy ASC-6P-72C-325-3BB | Solartech Energy ASC-6M-72-330-3BB | Solartech Energy ASC-6M-72B-330-3BB | Solartech Energy ASC-6M-72C-330-3BB | Solartech Energy ASC-6P-72-330-3BB | Solartech Energy ASC-6P-72B-330-3BB | Solartech Energy ASC-6P-72C-330-3BB | Solartech Energy ASC-6M-72-335-3BB | Solartech Energy ASC-6M-72B-335-3BB | Solartech Energy ASC-6M-72C-335-3BB | Solartech Power SPM190P | Solartech Power SPM195P | Solartech Power SPM200P | Solartech Power SPM205P | Solartech Power SPM210P | Solartech Power SPM220P | Solartech Power SPM225P | Solartech Power SPM230P | Solartech Power SPM235P | Solartech Power SPM240P | Solartech Renewables STR210 | Solartech Renewables STR215 | Solartech Renewables STR220 | Solartech Renewables STR225 | Solartech Renewables STR230 | SolarTech Universal STU-275 PERC | SolarTech Universal STU-280 PERC | SolarTech Universal PERCB-B-285 | SolarTech Universal PERCB-W-285 | SolarTech Universal STU-285 PERC | SolarTech Universal PERCB-B-290 | SolarTech Universal PERCB-W-290 | SolarTech Universal STU-290 PERC | SolarTech Universal HJTB-W-295 | SolarTech Universal PERCB-B-295 | SolarTech Universal PERCB-W-295 | SolarTech Universal STU-295 PERC | SolarTech Universal HJTB-W-300 | SolarTech Universal PERCB-B-300 | SolarTech Universal PERCB-W-300 | SolarTech Universal STU-300 PERC | SolarTech Universal STU-300-HJT | SolarTech Universal HJTB-W-305 | SolarTech Universal PERCB-B-305 | SolarTech Universal PERCB-W-305 | SolarTech Universal HJTB-W-310 | SolarTech Universal PERCB-B-310 | SolarTech Universal PERCB-W-310 | SolarTech Universal HJTB-W-315 | SolarTech Universal HJTB-W-320 | SolarTech Universal HJTB-W-325 | Solartechnics North America MP165Wp | Solartechnics North America MP170Wp | Solartechnics North America MP175Wp | Solartechnics North America MP180Wp | SolarWorld Americas Inc Sunmodule Bisun SWA 270 duo | SolarWorld Americas Inc Sunmodule Bisun SWA 270 duo black | SolarWorld Americas Inc Sunmodule Plus SWA 270 mono black | SolarWorld Americas Inc Sunmodule Protect SWA 270 mono | SolarWorld Americas Inc Sunmodule Bisun SWA 275 duo | SolarWorld Americas Inc Sunmodule Bisun SWA 275 duo black | SolarWorld Americas Inc Sunmodule Plus SWA 275 mono black | SolarWorld Americas Inc Sunmodule Bisun SWA 280 duo | SolarWorld Americas Inc Sunmodule Bisun SWA 280 duo black | SolarWorld Americas Inc Sunmodule Plus SWA 280 mono | SolarWorld Americas Inc Sunmodule Plus SWA 280 mono black | SolarWorld Americas Inc Sunmodule Plus SWA 280 mono black laminate | SolarWorld Americas Inc Sunmodule Protect SWA 280 mono | SolarWorld Americas Inc Sunmodule Plus SWA 285 mono | SolarWorld Americas Inc Sunmodule Plus SWA 285 mono black | SolarWorld Americas Inc Sunmodule Plus SWA 285 mono black laminate | SolarWorld Americas Inc Sunmodule Plus SWA 290 mono | SolarWorld Americas Inc Sunmodule Plus SWA 290 mono black | SolarWorld Americas Inc Sunmodule Plus SWA 290 mono black laminate | SolarWorld Americas Inc Sunmodule Protect SWA 290 mono | SolarWorld Americas Inc Sunmodule Plus SWA 295 mono | SolarWorld Americas Inc Sunmodule Plus SWA 295 mono black | SolarWorld Americas Inc Sunmodule Plus SWA 300 mono | SolarWorld Americas Inc Sunmodule Plus SWA 300 mono black | SolarWorld Americas Inc Sunmodule Plus SWA 305 mono | SolarWorld Americas Inc Sunmodule Plus SWA 305 mono black | SolarWorld Americas Inc Sunmodule Plus SWA 310 mono | SolarWorld Americas Inc Sunmodule Plus SWA 310 mono black | SolarWorld Americas Inc Sunmodule Plus SWA 315 mono | SolarWorld Americas Inc Sunmodule Bisun SWA 320 XL duo | SolarWorld Americas Inc Sunmodule SWA 320 XL mono | SolarWorld Americas Inc Sunmodule Bisun SWA 325 XL duo | SolarWorld Americas Inc Sunmodule SWA 325 XL mono | SolarWorld Americas Inc Sunmodule Bisun SWA 330 XL duo | SolarWorld Americas Inc Sunmodule SWA 330 XL mono black | SolarWorld Americas Inc Sunmodule SWA 335 XL mono | SolarWorld Americas Inc Sunmodule SWA 340 XL mono | SolarWorld Americas Inc Sunmodule SWA 340 XL mono black | SolarWorld Americas Inc Sunmodule SWA 345 XL mono | SolarWorld Americas Inc Sunmodule SWA 345 XL mono black | SolarWorld Americas Inc Sunmodule SWA 350 XL mono | SolarWorld Industries GmbH Sunmodule Plus SW 220 mono | SolarWorld 